simulink model "solar_pv_protected_c07_circuit"  (R2026b)
settings: Solver=VariableStepAuto
model workspace (MAT data in the model file):
  candidate_owner = 'pv_protection_integration_20261023_r01'
  solar_edit_metadata : object (value not decoded)
libraries: fl_lib x149, ee_lib x16, ltc4364demo_lib x3, batteryecm_lib x1, solarprotect_lib x1
(part 9 of 16)

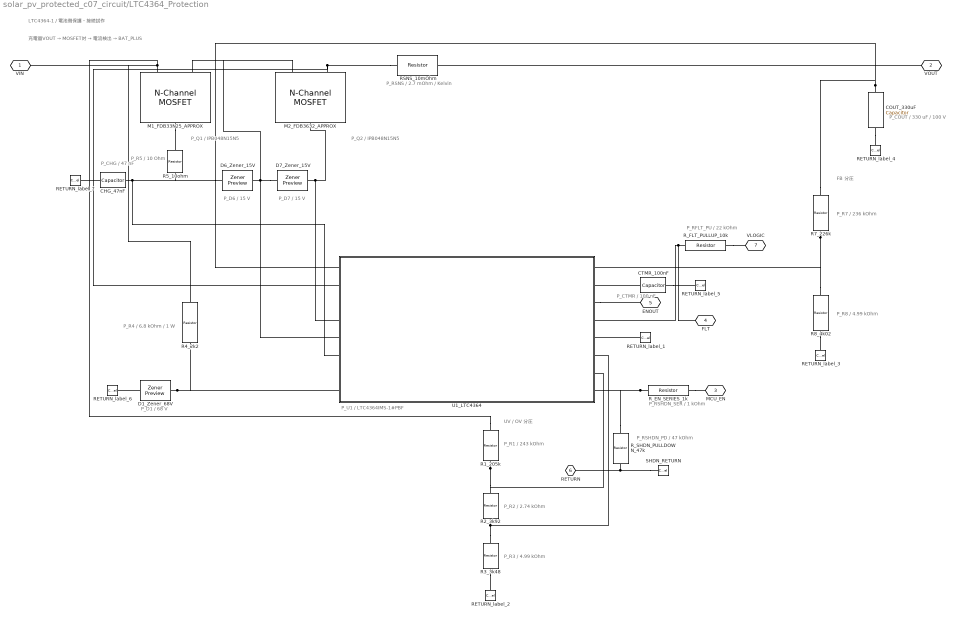
== system solar_pv_protected_c07_circuit/LTC4364_Protection ==
  note: FB 分圧
  note: UV / OV 分圧
  note: 充電器VOUT → MOSFET対 → 電流検出 → BAT_PLUS
  note: LTC4364-1 / 電池側保護・接続試作
  note: P_Q1 / IPB048N15N5
  note: P_Q2 / IPB048N15N5
  note: P_R4 / 6.8 kOhm / 1 W
  note: P_R5 / 10 Ohm
  note: P_RSNS / 2.7 mOhm / Kelvin
  note: P_CHG / 47 nF
  note: P_D6 / 15 V
  note: P_D7 / 15 V
  note: P_COUT / 330 uF / 100 V
  note: P_D1 / 68 V
  note: P_R1 / 243 kOhm
  note: P_R2 / 2.74 kOhm
  note: P_R3 / 4.99 kOhm
  note: P_R7 / 236 kOhm
  note: P_R8 / 4.99 kOhm
  note: P_CTMR / 100 nF
  note: P_RSHDN_SER / 1 kOhm
  note: P_RSHDN_PD / 47 kOhm
  note: P_RFLT_PU / 22 kOhm
  note: P_U1 / LTC4364IMS-1#PBF
  CHG_47nF : fl_lib/Electrical/Electrical Elements/Capacitor  Description=|  c=4.7e-08 F  r=0.01 Ohm  g=1e-10 1/Ohm  i_specify=off  i_priority=None  i=0 A  i_nominal_specify=off  i_nominal_value=1  i_nominal_unit=A  v_specify=off  v_priority=None  v=0 V  v_nominal_specify=off  v_nominal_value=1  v_nominal_unit=V  vc_specify=on  vc_priority=High  vc=0 V  vc_nominal_specify=off  vc_nominal_value=1  vc_nominal_unit=V
      | この回路での名前　　; P_CHG
      | 部品名　　　　　　　; CGA6P3C0G2E473J250AA
      | この回路での役割　　; 保護用MOSFET P_Q1のゲート電圧が立ち上がる速さを調整し、起動時の急な電流を抑える設計に使うコンデンサ。
      | ここでの動き　　　　; 保護ICがP_Q1を駆動する信号P_HGATEと共通GNDの間に47 nFを置き、その充放電によりゲート電圧の変化に時間を持たせる。P_Q1のゲートとソースの間へ直接付けた容量ではなく、起動と故障時の応答の両方に関わる。
      | 
      | 【詳しい働き・仕様・接続・確認の範囲】
      | 部品種別　　　　　　; 保護ゲートスルーレート用コンデンサ
      | 部品分類　　　　　　; 積層セラミックコンデンサ（MLCC）
      | 公称値　　　　　　　; 47 nF
      | 配置目的　　　　　　; HGATE–GND間へ置き、P_Q1起動時のゲート電圧変化と制御応答に関与させる。
      | 意図する動作　　　　; 47 nF。GND基準でありP_Q1のゲート–ソース容量そのものではない。容量変更は突入と故障応答を変える。
      | 端子と接続　　　　　; P P → P_HGATE、N N → GND
      | 部品の耐圧　　　　　; 250 V（既存メーカー資料照合記録の定格。回路全体の適合とは別。）
      | 公称値の公差　　　　; ±5%（既存部品資料の値）
      | 誘電体　　　　　　　; C0G
      | 部品資料の根拠　　　; TDKメーカーMLCC表で該当型番を確認した既存記録。動作時間とPCBでの使用条件は別確認。
      | モデルの範囲　　　　; Simscape標準コンデンサの集中定数表現。材質、DCバイアス、周波数依存ESR/ESL、寿命・温度特性を型番から自動再現するモデルではない。
      | モデル設定　　　　　; c=47 nF、r=10 mΩ、g=100 pS。これらは保存モデルの設定値であり、すべてが実部品の保証値という意味ではない。
      | 損失の扱い　　　　　; 保存モデルの直列抵抗rと実部品の周波数・温度依存ESRは区別する。容量値が一致しても損失・リプル電流・寿命の成立確認にはならない。
      | 確認の範囲　　　　　; 本説明は保存回路の部品情報・端子割当・既存設計意図を整理したもの。今回の説明更新によって新たな動作試験や実機検証を実施した意味ではない。
      | 設計記録　　　　　　; evaluation\component_annotations_20261022_r01\before_graph.json
      | evaluation\component_annotations_20261022_r01\before_metadata.json
      | evaluation\protection_capacitor_integration_20261021_r01\final_delivery\independent_readback\physical_bom.json
      | evaluation\protection_capacitor_integration_20261021_r01\capacitor_review\capacitor_inventory_after_c04.json
      | evaluation\protection_capacitor_integration_20261021_r01\protection_review\component_net_map.json
      | https://product.tdk.com/en/system/files/dam/doc/product/capacitor/ceramic/mlcc/catalog/mlcc_automotive_midvoltage_en.pdf
      | 
      | 【周波数・ノイズと配置の説明】
      | 周波数面の役割　　　; 保護用P_Q1の起動時ゲート電圧が変化する速さを調整し、突入と制御応答に関与する。
      | 対象周波数の目安　　; 主目的は特定周波数のノイズ除去ではなく時間応答の調整。47 nFとICのゲート駆動電流等がゲート電圧の変化速度に関係する。
      | ノイズの発生源　　　; LTC4364がHGATEを充放電するときの電流。ノイズ源に合わせたバイパス容量として選定したという意味ではない。
      | 他のコンデンサとの差; 電源バイパスと異なりHGATE–GND間に接続し、P_Q1のゲート–ソース間の容量そのものでもない。容量変更は起動と故障応答を変える。
      | 周波数説明の範囲　　; スルーレートと突入、保護応答は周辺素子とIC内部動作に依存する。47 nFだけから時間や安全性を保証しない。
      | 周波数説明の根拠　　; Analog Devices：LTC4364-1/LTC4364-2 datasheet
      | https://www.analog.com/media/en/technical-documentation/data-sheets/ltc4364-1-4364-2.pdf
      | 
      | 【この説明欄の略語・記号】
      | 用語1　　　　　　　 ; MLCC：Multilayer Ceramic Capacitor（積層セラミックコンデンサ）。薄いセラミック誘電体と電極を重ねたコンデンサ。対象周波数は容量・実装・寄生成分で変わるため、MLCCという分類だけでは決めない。
      | 用語2　　　　　　　 ; ESR：Equivalent Series Resistance（等価直列抵抗）。コンデンサの損失を直列抵抗で表した量。周波数・温度で変わり、損失とリプル電圧に関係する。
      | 用語3　　　　　　　 ; ESL：Equivalent Series Inductance（等価直列インダクタンス）。端子や電極などの寄生インダクタンスを表す。高い周波数ではバイパス効果を制限する。
      | 用語4　　　　　　　 ; DC：Direct Current（直流）。ここでは直流電源または直流成分。DCバイアスはコンデンサに重なる直流電圧を指す。
      | 用語5　　　　　　　 ; C0G：温度補償系セラミックコンデンサの温度特性記号。英語の頭文字ではなく分類コード。−55〜+125 ℃で容量の温度係数が0±30 ppm/℃の特性を表す。ppmはparts per million（100万分の1）で、30 ppm/℃は1 ℃当たり0.003%に相当する。
      | 用語6　　　　　　　 ; IC：Integrated Circuit（集積回路）。複数の電子素子と機能を小さな半導体チップに集積した部品。
      | 用語7　　　　　　　 ; PWM：Pulse Width Modulation（パルス幅変調）。周期に対するON時間の割合を変えて、スイッチの平均的な電力伝達を調整する方式。
      | 用語8　　　　　　　 ; MOSFET：Metal-Oxide-Semiconductor Field-Effect Transistor（金属・酸化膜・半導体構造の電界効果トランジスタ）。ゲートとソースの電圧でドレインとソースの導通を制御する素子。N-MOSはNチャネル型を表す。
      | 用語9　　　　　　　 ; PCB：Printed Circuit Board（プリント配線板）。部品を実装し、銅配線で接続する基板。
      | 用語10　　　　　　　; GND：Ground（回路の基準電位・電流帰路）。この図の共通基準。保護接地や大地への接続を意味するとは限らない。
      | 用語11　　　　　　　; HGATE/DGATE：LTC4364の二つの外付けMOSFETゲート駆動出力。HGATEは主に電圧・電流制限側のP_Q1、DGATEは理想ダイオード／逆流防止側のP_Q2を駆動する。主電力段の上下PWMとは別の仕組み。
  COUT_330uF : fl_lib/Electrical/Electrical Elements/Capacitor  Description=|  c=330e-6 F  r=0.01 Ohm  g=1e-10 1/Ohm  i_specify=off  i_priority=None  i=0 A  i_nominal_specify=off  i_nominal_value=1  i_nominal_unit=A  v_specify=off  v_priority=None  v=0 V  v_nominal_specify=off  v_nominal_value=1  v_nominal_unit=V  vc_specify=off  vc_priority=High  vc=0 V  vc_nominal_specify=off  vc_nominal_value=1  vc_nominal_unit=V
      | この回路での名前　　; P_COUT
      | 部品名　　　　　　　; 100ZLH330MEFC12.5X35
      | この回路での役割　　; 保護回路を通ったバッテリー側に電荷を蓄え、その場所の電圧・電流の変化を受け止めるためのコンデンサ。
      | ここでの動き　　　　; 保護出力BAT_PLUSと共通GNDの間に330 µFを置く。保護が遮断してもバッテリー側に残るため、保護前のC13〜C16と常に同じ働きをする並列容量としては扱わない。
      | 
      | 【詳しい働き・仕様・接続・確認の範囲】
      | 部品種別　　　　　　; 保護出力側バルクコンデンサ
      | 部品分類　　　　　　; アルミ電解コンデンサ（有極性）
      | 公称値　　　　　　　; 330 µF
      | 配置目的　　　　　　; BAT_PLUS–GND間へ配置し、保護回路下流側の局所的な電荷を受け持つ。
      | 意図する動作　　　　; 上流VOUTのC13〜C16とは保護OFF時に別ノードとなり、同じ目的の重複部品ではない。330 µFの実効容量・リプル・熱の適合は別確認。
      | 端子と接続　　　　　; P P → BAT_PLUS、N N → GND
      | 部品の耐圧　　　　　; 100 V（既存メーカー資料照合記録の定格。回路全体の適合とは別。）
      | 公称値の公差　　　　; ±20%（既存部品資料の値）
      | 部品資料の根拠　　　; Rubycon ZLHメーカー表の100 V・330 µF・12.5×35 mmと品番構成に基づく既存照合記録。43 mΩは100 kHzインピーダンスの上限であり、全周波数の一定ESRではない。
      | モデルの範囲　　　　; Simscape標準コンデンサの集中定数表現。材質、DCバイアス、周波数依存ESR/ESL、寿命・温度特性を型番から自動再現するモデルではない。
      | モデル設定　　　　　; c=330 µF、r=10 mΩ、g=100 pS。これらは保存モデルの設定値であり、すべてが実部品の保証値という意味ではない。
      | 損失の扱い　　　　　; 保存モデルの直列抵抗rと実部品の周波数・温度依存ESRは区別する。容量値が一致しても損失・リプル電流・寿命の成立確認にはならない。
      | 確認の範囲　　　　　; 本説明は保存回路の部品情報・端子割当・既存設計意図を整理したもの。今回の説明更新によって新たな動作試験や実機検証を実施した意味ではない。
      | 設計記録　　　　　　; evaluation\component_annotations_20261022_r01\before_graph.json
      | evaluation\component_annotations_20261022_r01\before_metadata.json
      | evaluation\protection_capacitor_integration_20261021_r01\final_delivery\independent_readback\physical_bom.json
      | evaluation\protection_capacitor_integration_20261021_r01\capacitor_review\capacitor_inventory_after_c04.json
      | evaluation\protection_capacitor_integration_20261021_r01\protection_review\component_net_map.json
      | https://www.rubycon.co.jp/wp-content/uploads/catalog-aluminum/ZLH.pdf
      | 
      | 【周波数・ノイズと配置の説明】
      | 周波数面の役割　　　; 保護回路の下流BAT_PLUS側に局所的な電荷を蓄える。
      | 対象周波数の目安　　; 起動/遮断/負荷変化の過渡と、通電時に上流から届くリプルが対象。具体的な有効帯域は回路と実装に依存する。
      | ノイズの発生源　　　; 保護MOSFETをオン・オフする過渡、配線を通じたバッテリー電流変化、保護が導通中の上流降圧回路のリプル。
      | 他のコンデンサとの差; C13/C14の上流VOUT側と異なり、遮断中もBAT_PLUS側に残る330 µF電解。上流の大容量と単純に並列合算できない。
      | 周波数説明の範囲　　; 狙うノイズの周波数と、この部品が実装後に有効な周波数範囲は別である。実効容量、等価直列抵抗、等価直列インダクタンス、配線を含む自己共振で変わるため、型番名や公称容量だけから有効帯域の上限を断定しない。
      | 周波数説明の根拠　　; Analog Devices：LTC4364-1/LTC4364-2 datasheet
      | https://www.analog.com/media/en/technical-documentation/data-sheets/ltc4364-1-4364-2.pdf
      | 村田製作所：コンデンサのインピーダンス・ESRと周波数の関係
      | https://article.murata.com/en-global/article/impedance-esr-frequency-characteristics-in-capacitors
      | 
      | 【この説明欄の略語・記号】
      | 用語1　　　　　　　 ; ESR：Equivalent Series Resistance（等価直列抵抗）。コンデンサの損失を直列抵抗で表した量。周波数・温度で変わり、損失とリプル電圧に関係する。
      | 用語2　　　　　　　 ; ESL：Equivalent Series Inductance（等価直列インダクタンス）。端子や電極などの寄生インダクタンスを表す。高い周波数ではバイパス効果を制限する。
      | 用語3　　　　　　　 ; DC：Direct Current（直流）。ここでは直流電源または直流成分。DCバイアスはコンデンサに重なる直流電圧を指す。
      | 用語4　　　　　　　 ; MOSFET：Metal-Oxide-Semiconductor Field-Effect Transistor（金属・酸化膜・半導体構造の電界効果トランジスタ）。ゲートとソースの電圧でドレインとソースの導通を制御する素子。N-MOSはNチャネル型を表す。
      | 用語5　　　　　　　 ; GND：Ground（回路の基準電位・電流帰路）。この図の共通基準。保護接地や大地への接続を意味するとは限らない。
      | 用語6　　　　　　　 ; VIN/VOUT：入力電圧・出力電圧を表す端子／ネット名。INは入力、OUTは出力。電源変換器の電力端子なのか、検出用端子なのかは対象部品によって異なるため、端子と接続の説明に従う。
  CTMR_100nF : fl_lib/Electrical/Electrical Elements/Capacitor  Description=|  c=1e-07 F  r=0.01 Ohm  g=1e-10 1/Ohm  i_specify=off  i_priority=None  i=0 A  i_nominal_specify=off  i_nominal_value=1  i_nominal_unit=A  v_specify=off  v_priority=None  v=0 V  v_nominal_specify=off  v_nominal_value=1  v_nominal_unit=V  vc_specify=on  vc_priority=High  vc=0 V  vc_nominal_specify=off  vc_nominal_value=1  vc_nominal_unit=V
      | この回路での名前　　; P_CTMR
      | 部品名　　　　　　　; CGA5L2C0G1H104J160AE
      | この回路での役割　　; 保護ICが異常の継続時間を判断し、遮断へ移るタイミングを決めるためのコンデンサ。
      | ここでの動き　　　　; 保護ICの時間設定信号P_TMRと共通GNDの間に100 nFを置き、内部電流による充放電を時間の判断に使う。遮断までの時間は容量だけでなく、故障状態やIC内部の電流・判定電圧にも依存する。
      | 
      | 【詳しい働き・仕様・接続・確認の範囲】
      | 部品種別　　　　　　; 保護故障タイマ用コンデンサ
      | 部品分類　　　　　　; 積層セラミックコンデンサ（MLCC）
      | 公称値　　　　　　　; 100 nF
      | 配置目的　　　　　　; TMR–GND間に置き、故障継続時間の積算・遮断タイミングへ関与させる。
      | 意図する動作　　　　; 100 nF。タイマ電流と比較しきい値にも依存し、公称容量だけで遮断時間は一意に保証されない。
      | 端子と接続　　　　　; P P → P_TMR、N N → GND
      | 部品の耐圧　　　　　; 50 V（既存メーカー資料照合記録の定格。回路全体の適合とは別。）
      | 公称値の公差　　　　; ±5%（既存部品資料の値）
      | 誘電体　　　　　　　; C0G
      | 部品資料の根拠　　　; TDKメーカーMLCC表で該当型番を確認した既存記録。動作時間とPCBでの使用条件は別確認。
      | モデルの範囲　　　　; Simscape標準コンデンサの集中定数表現。材質、DCバイアス、周波数依存ESR/ESL、寿命・温度特性を型番から自動再現するモデルではない。
      | モデル設定　　　　　; c=100 nF、r=10 mΩ、g=100 pS。これらは保存モデルの設定値であり、すべてが実部品の保証値という意味ではない。
      | 損失の扱い　　　　　; 保存モデルの直列抵抗rと実部品の周波数・温度依存ESRは区別する。容量値が一致しても損失・リプル電流・寿命の成立確認にはならない。
      | 確認の範囲　　　　　; 本説明は保存回路の部品情報・端子割当・既存設計意図を整理したもの。今回の説明更新によって新たな動作試験や実機検証を実施した意味ではない。
      | 設計記録　　　　　　; evaluation\component_annotations_20261022_r01\before_graph.json
      | evaluation\component_annotations_20261022_r01\before_metadata.json
      | evaluation\protection_capacitor_integration_20261021_r01\final_delivery\independent_readback\physical_bom.json
      | evaluation\protection_capacitor_integration_20261021_r01\capacitor_review\capacitor_inventory_after_c04.json
      | evaluation\protection_capacitor_integration_20261021_r01\protection_review\component_net_map.json
      | https://product.tdk.com/system/files/dam/doc/product/capacitor/ceramic/mlcc/catalog/mlcc_automotive_soft_en.pdf
      | 
      | 【周波数・ノイズと配置の説明】
      | 周波数面の役割　　　; 故障がどれだけ継続したかを電荷として積算し、遮断までの時間に関与するタイマ容量。
      | 対象周波数の目安　　; 主目的はノイズの周波数選別ではない。容量、IC内部の充放電電流、比較しきい値から時間が決まるため、「100 nFの高周波ノイズ用」とは説明しない。
      | ノイズの発生源　　　; 想定する入力はLTC4364の故障状態に応じたタイマ充放電。測定したノイズ周波数をこの部品へ割り当ててはいない。
      | 他のコンデンサとの差; 同じ100 nFのC17/C36等は電源バイパス。本品は時間設定であり、部品種が同じでも役割は異なる。
      | 周波数説明の範囲　　; 遮断時間は型番の内部電流・しきい値、故障条件、初期状態も含めて評価する。公称容量だけで保証しない。
      | 周波数説明の根拠　　; Analog Devices：LTC4364-1/LTC4364-2 datasheet
      | https://www.analog.com/media/en/technical-documentation/data-sheets/ltc4364-1-4364-2.pdf
      | 
      | 【この説明欄の略語・記号】
      | 用語1　　　　　　　 ; MLCC：Multilayer Ceramic Capacitor（積層セラミックコンデンサ）。薄いセラミック誘電体と電極を重ねたコンデンサ。対象周波数は容量・実装・寄生成分で変わるため、MLCCという分類だけでは決めない。
      | 用語2　　　　　　　 ; ESR：Equivalent Series Resistance（等価直列抵抗）。コンデンサの損失を直列抵抗で表した量。周波数・温度で変わり、損失とリプル電圧に関係する。
      | 用語3　　　　　　　 ; ESL：Equivalent Series Inductance（等価直列インダクタンス）。端子や電極などの寄生インダクタンスを表す。高い周波数ではバイパス効果を制限する。
      | 用語4　　　　　　　 ; DC：Direct Current（直流）。ここでは直流電源または直流成分。DCバイアスはコンデンサに重なる直流電圧を指す。
      | 用語5　　　　　　　 ; C0G：温度補償系セラミックコンデンサの温度特性記号。英語の頭文字ではなく分類コード。−55〜+125 ℃で容量の温度係数が0±30 ppm/℃の特性を表す。ppmはparts per million（100万分の1）で、30 ppm/℃は1 ℃当たり0.003%に相当する。
      | 用語6　　　　　　　 ; IC：Integrated Circuit（集積回路）。複数の電子素子と機能を小さな半導体チップに集積した部品。
      | 用語7　　　　　　　 ; PCB：Printed Circuit Board（プリント配線板）。部品を実装し、銅配線で接続する基板。
      | 用語8　　　　　　　 ; GND：Ground（回路の基準電位・電流帰路）。この図の共通基準。保護接地や大地への接続を意味するとは限らない。
      | 用語9　　　　　　　 ; TMR：Timer（時間設定端子）。LTC4364では外付けコンデンサにより故障継続時間の判定などに関係する時間を設定する。
  D1_Zener_68V : ltc4364demo_lib/Zener Preview  Description=|  Vz=68 V  Rz=5 Ohm  Vf=0.7 V  Rf=1 Ohm  i_specify=off  i_priority=None  i=0 A  i_nominal_specify=off  i_nominal_value=1  i_nominal_unit=A
      | この回路での名前　　; P_D1
      | 部品名　　　　　　　; CMZ5945B TR13 PBFREE
      | この回路での役割　　; 保護IC P_U1の電源電圧が上がりすぎるのを抑えるダイオード。
      | ここでの動き　　　　; 保護ICの電源とGNDの間に接続し、電圧が上がったときに電流を逃がす。直列抵抗P_R4と組み合わせて使う。
      | 
      | 【詳しい働き・仕様・接続・確認の範囲】
      | 部品種別　　　　　　; 保護IC電源クランプ・ツェナー
      | 公称値　　　　　　　; 68 V
      | 配置目的　　　　　　; P_VCC–GND間でLTC4364の電源電圧上昇を抑える。
      | 意図する動作　　　　; 公称68 V。P_R4と組み合わせる。クランプ公差・電流依存・持続損失・PCB放熱の成立は別確認。
      | 端子と接続　　　　　; A A → GND、K K → P_VCC
      | 部品資料の根拠　　　; Central Semiconductor公式製品情報のCMZ5945B TR13と、鉛フリー接尾辞PBFREEの既存確認記録。
      | モデルの範囲　　　　; Simscapeダイオード素子による近似。順方向損失、漏れ、温度依存、逆回復・接合容量の型番固有特性を完全に再現するものではない。
      | モデル設定　　　　　; Vf=700 mV、Vz=68 V。これらは保存モデルの設定値であり、すべてが実部品の保証値という意味ではない。
      | 確認の範囲　　　　　; 本説明は保存回路の部品情報・端子割当・既存設計意図を整理したもの。今回の説明更新によって新たな動作試験や実機検証を実施した意味ではない。
      | 設計記録　　　　　　; evaluation\component_annotations_20261022_r01\before_graph.json
      | evaluation\component_annotations_20261022_r01\before_metadata.json
      | evaluation\protection_capacitor_integration_20261021_r01\final_delivery\independent_readback\physical_bom.json
      | evaluation\protection_capacitor_integration_20261021_r01\protection_review\component_net_map.json
      | 
      | 【この説明欄の略語・記号】
      | 用語1　　　　　　　 ; IC：Integrated Circuit（集積回路）。複数の電子素子と機能を小さな半導体チップに集積した部品。
      | 用語2　　　　　　　 ; MOSFET：Metal-Oxide-Semiconductor Field-Effect Transistor（金属・酸化膜・半導体構造の電界効果トランジスタ）。ゲートとソースの電圧でドレインとソースの導通を制御する素子。N-MOSはNチャネル型を表す。
      | 用語3　　　　　　　 ; Vf：Forward Voltage（順方向電圧）。ダイオードが順方向に電流を流すときの電圧降下。電流・温度で変わる。
      | 用語4　　　　　　　 ; Vz：Zener Voltage（ツェナー電圧）。ツェナーダイオードの逆方向での電圧制限に関係する値。
      | 用語5　　　　　　　 ; PCB：Printed Circuit Board（プリント配線板）。部品を実装し、銅配線で接続する基板。
      | 用語6　　　　　　　 ; GND：Ground（回路の基準電位・電流帰路）。この図の共通基準。保護接地や大地への接続を意味するとは限らない。
      | 用語7　　　　　　　 ; VCC/VDD/VEE/VS：ICの電源端子名。文字の歴史的な由来を現在の接続機能へ当てはめない。現回路のVEEはU8/U10では浮動基準SW、U9ではGND。各電圧・基準は端子と接続を参照する。
      | 用語8　　　　　　　 ; SW：Switching Node（スイッチング点）。主電力段の上下MOSFETとL1がつながる、電圧が高速に切り替わる点。GNDとは別電位。
  D6_Zener_15V : ltc4364demo_lib/Zener Preview  Description=|  Vz=15 V  Rz=5 Ohm  Vf=0.7 V  Rf=1 Ohm  i_specify=off  i_priority=None  i=0 A  i_nominal_specify=off  i_nominal_value=1  i_nominal_unit=A
      | この回路での名前　　; P_D6
      | 部品名　　　　　　　; DDZ9702T
      | この回路での役割　　; 保護用MOSFET P_Q1を駆動する電圧が、ソースに対して高くなりすぎるのを抑えるダイオード。
      | ここでの動き　　　　; 保護ICのゲート駆動出力HGATEと、P_Q1/P_Q2共通のソース点の間に置く。共通GNDに対する電圧を抑える部品ではない。
      | 
      | 【詳しい働き・仕様・接続・確認の範囲】
      | 部品種別　　　　　　; HGATE–共通ソース間ツェナー
      | 公称値　　　　　　　; 15 V
      | 配置目的　　　　　　; HGATEとP_SOURCE間でP_Q1側のゲート電圧上昇を抑える。
      | 意図する動作　　　　; 公称15 V。P_SOURCEはGNDではない。P_R5よりIC側に配置されたクランプ。
      | 端子と接続　　　　　; A A → P_SOURCE、K K → P_HGATE
      | 部品資料の根拠　　　; Diodes Incorporated DDZ96xxT/DDZ97xxTデータシートに公称15 VのDDZ9702Tを確認した既存記録。梱包接尾辞とパルス電力の適合は未確定。
      | モデルの範囲　　　　; Simscapeダイオード素子による近似。順方向損失、漏れ、温度依存、逆回復・接合容量の型番固有特性を完全に再現するものではない。
      | モデル設定　　　　　; Vf=700 mV、Vz=15 V。これらは保存モデルの設定値であり、すべてが実部品の保証値という意味ではない。
      | 確認の範囲　　　　　; 本説明は保存回路の部品情報・端子割当・既存設計意図を整理したもの。今回の説明更新によって新たな動作試験や実機検証を実施した意味ではない。
      | 設計記録　　　　　　; evaluation\component_annotations_20261022_r01\before_graph.json
      | evaluation\component_annotations_20261022_r01\before_metadata.json
      | evaluation\protection_capacitor_integration_20261021_r01\final_delivery\independent_readback\physical_bom.json
      | evaluation\protection_capacitor_integration_20261021_r01\protection_review\component_net_map.json
      | 
      | 【この説明欄の略語・記号】
      | 用語1　　　　　　　 ; IC：Integrated Circuit（集積回路）。複数の電子素子と機能を小さな半導体チップに集積した部品。
      | 用語2　　　　　　　 ; PWM：Pulse Width Modulation（パルス幅変調）。周期に対するON時間の割合を変えて、スイッチの平均的な電力伝達を調整する方式。
      | 用語3　　　　　　　 ; MOSFET：Metal-Oxide-Semiconductor Field-Effect Transistor（金属・酸化膜・半導体構造の電界効果トランジスタ）。ゲートとソースの電圧でドレインとソースの導通を制御する素子。N-MOSはNチャネル型を表す。
      | 用語4　　　　　　　 ; Vf：Forward Voltage（順方向電圧）。ダイオードが順方向に電流を流すときの電圧降下。電流・温度で変わる。
      | 用語5　　　　　　　 ; Vz：Zener Voltage（ツェナー電圧）。ツェナーダイオードの逆方向での電圧制限に関係する値。
      | 用語6　　　　　　　 ; GND：Ground（回路の基準電位・電流帰路）。この図の共通基準。保護接地や大地への接続を意味するとは限らない。
      | 用語7　　　　　　　 ; HGATE/DGATE：LTC4364の二つの外付けMOSFETゲート駆動出力。HGATEは主に電圧・電流制限側のP_Q1、DGATEは理想ダイオード／逆流防止側のP_Q2を駆動する。主電力段の上下PWMとは別の仕組み。
  D7_Zener_15V : ltc4364demo_lib/Zener Preview  Description=|  Vz=15 V  Rz=5 Ohm  Vf=0.7 V  Rf=1 Ohm  i_specify=off  i_priority=None  i=0 A  i_nominal_specify=off  i_nominal_value=1  i_nominal_unit=A
      | この回路での名前　　; P_D7
      | 部品名　　　　　　　; DDZ9702T
      | この回路での役割　　; 逆流防止用MOSFET P_Q2のゲート電圧が、ソースに対して高くなりすぎるのを抑えるダイオード。
      | ここでの動き　　　　; 保護ICのゲート駆動出力DGATEと、P_Q1/P_Q2共通のソース点の間に置く。
      | 
      | 【詳しい働き・仕様・接続・確認の範囲】
      | 部品種別　　　　　　; DGATE–共通ソース間ツェナー
      | 公称値　　　　　　　; 15 V
      | 配置目的　　　　　　; DGATEとP_SOURCE間でP_Q2のゲート電圧上昇を抑える。
      | 意図する動作　　　　; 公称15 V。動的クランプとパルス電力は未適合確認。
      | 端子と接続　　　　　; A A → P_SOURCE、K K → P_DGATE
      | 部品資料の根拠　　　; Diodes Incorporated DDZ96xxT/DDZ97xxTデータシートに公称15 VのDDZ9702Tを確認した既存記録。梱包接尾辞とパルス電力の適合は未確定。
      | モデルの範囲　　　　; Simscapeダイオード素子による近似。順方向損失、漏れ、温度依存、逆回復・接合容量の型番固有特性を完全に再現するものではない。
      | モデル設定　　　　　; Vf=700 mV、Vz=15 V。これらは保存モデルの設定値であり、すべてが実部品の保証値という意味ではない。
      | 確認の範囲　　　　　; 本説明は保存回路の部品情報・端子割当・既存設計意図を整理したもの。今回の説明更新によって新たな動作試験や実機検証を実施した意味ではない。
      | 設計記録　　　　　　; evaluation\component_annotations_20261022_r01\before_graph.json
      | evaluation\component_annotations_20261022_r01\before_metadata.json
      | evaluation\protection_capacitor_integration_20261021_r01\final_delivery\independent_readback\physical_bom.json
      | evaluation\protection_capacitor_integration_20261021_r01\protection_review\component_net_map.json
      | 
      | 【この説明欄の略語・記号】
      | 用語1　　　　　　　 ; PWM：Pulse Width Modulation（パルス幅変調）。周期に対するON時間の割合を変えて、スイッチの平均的な電力伝達を調整する方式。
      | 用語2　　　　　　　 ; MOSFET：Metal-Oxide-Semiconductor Field-Effect Transistor（金属・酸化膜・半導体構造の電界効果トランジスタ）。ゲートとソースの電圧でドレインとソースの導通を制御する素子。N-MOSはNチャネル型を表す。
      | 用語3　　　　　　　 ; Vf：Forward Voltage（順方向電圧）。ダイオードが順方向に電流を流すときの電圧降下。電流・温度で変わる。
      | 用語4　　　　　　　 ; Vz：Zener Voltage（ツェナー電圧）。ツェナーダイオードの逆方向での電圧制限に関係する値。
      | 用語5　　　　　　　 ; HGATE/DGATE：LTC4364の二つの外付けMOSFETゲート駆動出力。HGATEは主に電圧・電流制限側のP_Q1、DGATEは理想ダイオード／逆流防止側のP_Q2を駆動する。主電力段の上下PWMとは別の仕組み。
  M1_FDB33N25_APPROX : ee_lib/Semiconductors & Converters/N-Channel MOSFET  Description=|  paramTerminal=ee.enum.mosfet.numberOfTerminals.three  parameterization=ee.enum.mosfet.parameterization.datasheet  Beta=5.0 A/V^2  Rds=0.0048 Ohm  Id=4 A  Vgs=10 V  Vth=4.1 V  Vth0=1.7 V  lam=0 1/V  gamma_vth=0.5 V^(1/2)  phib=0.5 V  Vth1=1.9071 V  Vbs1=-1 V  Vth2=2.066 V  Vbs2=-2 V  Tmeas=25 degC  Vgs_vec=[-1, -.5, 2, 3, 4, 5] V  Vds_vec=[0, 2, 4, 8, 12, 16, 20] V  Vbs_vec=[0, -4, -6, -12] V  T_vec=[25, 125] degC  Vth_vec=[.4, 1.2, 1.4, 1.45] V  Vth_mat=[.4, .35; 1.2, 1.15; 1.4, 1.35; 1.45, 1.4] V  Ids_mat=[0, 0, 0, 0, 0, 0, 0; 0, 0, 0, 0, 0, 0, 0; 0, .003, .0038, .0043, .0046, .0048, .0049; 0, .0055, .008, .009, .0095, .01, .0101; 0, .0115, .016, .018, .019, .0195, .02; 0, .0152, .0225, .0265, .028, .0295, .03] A  Ids_mat0=[0, 0, 0, 0, 0, 0, 0; 0, 0, 0, 0, 0, 0, 0; 0, .003, .0038, .0043, .0046, .0048, .0049; 0, .0055, .008, .009, .0095, .01, .0101; 0, .0115, .016, .018, .019, .0195, .02; 0, .0152, .0225, .0265, .028, .0295, .03] A  Ids_mat_3D=zeros(6, 7, 2) A  Ids_mat_3D0=zeros(6, 7, 2) A  IV_table_symmetry=ee.enum.mosfet.symmetricNIV.no  RS=0.0001 Ohm  RD=0.0001 Ohm  RB=0.001 Ohm  LeadRs=0 Ohm  LeadRd=0 Ohm  LeadRg=25 Ohm  LeadRb=0 Ohm  LS=0 nH  LD=0 nH  LG=0 nH  LB=0 nH  C_param=ee.enum.mosfet.capacitanceParam.fixedciss  C_GS=270 pF  C_GD=80 pF  C_GB=0 pF  C_DS=0 pF  C_iss=290e-12 F  C_rss=13e-12 F  C_oss=1400e-12 F  C_iss_vec=[720, 700, 590, 470, 390, 310] pF  C_rss_vec=[450, 400, 300, 190, 95, 55] pF  C_oss_vec=[900, 810, 690, 420, 270, 170] pF  C_GS_vec=[270, 300, 290, 280, 295, 255] pF  C_GD_vec=[450, 400, 300, 190, 95, 55] pF  C_GB_vec=[270, 300, 290, 280, 295, 255] pF  C_Vgs_vec=0 V  C_DS_vec=[450, 410, 390, 230, 175, 115] pF  C_Vds_vec=[.1, .3, 1, 3, 10, 30] V  V_GS_for_cap_data=0 V  charge_linearity_param=ee.enum.mosfet.cgdLinearity.constant  C_OX=200 pF  V_C_OX=-0.5 V  charge_linearity_param_vgb=ee.enum.mosfet.cgbLinearity.instantly  charge_linearity_param_with_vgb=ee.enum.mosfet.cgbLinearityWithSeparateCgb.instantly  Di_param=ee.enum.mosfet.diodeParam.exponential  IsDiode=1e-9 A  Vbi=0.6 V  n=1.5  Cj0Diode=0 pF  TT=0 s  Tmeas_dio=25 degC  TableTypeNoT=ee.enum.mosfet.tableType.IfMat  TableType=ee.enum.diode.tableType.IfMat  IfVec=[.07, .12, .19, 1.75, 4.24, 7.32, 11.2] A  IfMat=[.07, .12, .19, 1.75, 4.24, 7.32, 11.2; .16, .3, .72, 2.14, 4.02, 6.35, 9.12] A  VfVecV=[.9, 1.15, 1.25, 1.5, 1.75, 2.17, 2.6, 2.85] V  VfMatV=[.9, 1.15, 1.25, 1.5, 1.75, 2.17, 2.6, 2.85; .58, .68, .75, 1.1, 1.38, 1.77, 2.27, 2.7] V  TjVec=[25, 125] degC  VfVec=[.5, .7, .9, 1.3, 1.7, 2.1, 2.5] V  IfVecV=[.1, .2, .5, 1, 2, 4, 7, 10] A  diode_Goff=1e-12 1/Ohm  prmDatasheet=ee.enum.temperatureParameterization.none  prmEquCoeff=ee.enum.temperatureParameterization.none  dVth_dT=-6 mV/K  dVth0_dT=-6 mV/K  Rds_T2=0.037 Ohm  BEXDatasheet=-1.5  BEXEquCoeff=-1.5  etaisDatasheet=3  etaisEquCoeff=3  Tmeas2=125 degC  etaisTabulated=3  TdeviceDatasheet=25 degC  TdeviceEquCoeff=25 degC  TdeviceTabulated=25 degC  i_g_specify=off  i_g_priority=None  i_g=0 A  i_g_nominal_specify=off  i_g_nominal_value=1  i_g_nominal_unit=A  i_d_specify=off  i_d_priority=None  i_d=0 A  i_d_nominal_specify=off  i_d_nominal_value=1  i_d_nominal_unit=A  i_b_specify=off  i_b_priority=None  i_b=0 A  i_b_nominal_specify=off  i_b_nominal_value=1  i_b_nominal_unit=A  voltage_gs_specify=off  voltage_gs_priority=None  voltage_gs=0 V  voltage_gs_nominal_specify=off  voltage_gs_nominal_value=1  voltage_gs_nominal_unit=V  voltage_ds_specify=off  voltage_ds_priority=None  voltage_ds=0 V  voltage_ds_nominal_specify=off  voltage_ds_nominal_value=1  voltage_ds_nominal_unit=V  voltage_bs_specify=off  voltage_bs_priority=None  voltage_bs=0 V  voltage_bs_nominal_specify=off  voltage_bs_nominal_value=1  voltage_bs_nominal_unit=V  v_Cgs_specify=off  v_Cgs_priority=High  v_Cgs=0 V  v_Cgs_nominal_specify=off  v_Cgs_nominal_value=1  v_Cgs_nominal_unit=V  v_Cds_specify=off  v_Cds_priority=High  v_Cds=0 V  v_Cds_nominal_specify=off  v_Cds_nominal_value=1  v_Cds_nominal_unit=V  v_Cbs_specify=off  v_Cbs_priority=High  v_Cbs=0 V  v_Cbs_nominal_specify=off  v_Cbs_nominal_value=1  v_Cbs_nominal_unit=V  thermal_network_parameterization=ee.enum.thermalNetworkTopology.junctionCase  Rth=[0, 10] K/W  Rth_Cauer=[1, 3, 10] K/W  Rth_Foster=[.08, .14, .22, .16] K/W  thermal_mass_parameterization=ee.enum.thermalNetwork.timeconstant  thermal_mass=[0, 1] J/K  thermal_mass_Cauer=[.1, .3, 1] J/K  thermal_mass_Foster=[.001, .005, .05, .5] J/K  thermal_time_constant=[0, 10] s  thermal_time_constant_Cauer=[1, 3, 10] s  thermal_time_constant_Foster=[7e-05, .0007, .01, .08] s  thermal_mass_initial_temperatures=[25, 25] degC  thermal_mass_initial_temperatures_Cauer=[25, 25, 25] degC  Tvec_initial_Foster=[25, 25, 25, 25] degC  betaref=18 A/V^2  Vfbref=-1.1 V  gamma=3.5 V^(1/2)  phib2ref=1 V  thesatref=0.4 1/V  alpha=0  Vp=5e-2 V  thesrref=0 1/V  m=8  Tref=25 degC  Rsref=2e-3 Ohm  Rdref=0.17 Ohm  Rgref=8.4 Ohm  Rbref=2e-3 Ohm  Cox=1500 pF  Cgso=100 pF  Cgdo=14 pF  Isref=5.2e-13 A  Cj0=480 pF  Tprm=ee.enum.temperatureParameterization.none  etabet=1.3  Stvfb=5e-4 V/K  Stphib=-8.5e-4 V/K  etasat=1.04  etasr=0.65  etar=0.95  etais=3  Tsim=25 degC  Ig_specify=off  Ig_priority=None  Ig=0 A  Ig_nominal_specify=off  Ig_nominal_value=1  Ig_nominal_unit=nA  Ids_specify=off  Ids_priority=None  Ids=0 A  Ids_nominal_specify=off  Ids_nominal_value=1  Ids_nominal_unit=A  Ib_specify=off  Ib_priority=None  Ib=0 A  Ib_nominal_specify=off  Ib_nominal_value=1  Ib_nominal_unit=uA  V_gs_specify=off  V_gs_priority=None  V_gs=0 V  V_gs_nominal_specify=off  V_gs_nominal_value=1  V_gs_nominal_unit=V  V_ds_specify=off  V_ds_priority=None  V_ds=0 V  V_ds_nominal_specify=off  V_ds_nominal_value=1  V_ds_nominal_unit=V  V_bs_specify=off  V_bs_priority=None  V_bs=0 V  V_bs_nominal_specify=off  V_bs_nominal_value=1  V_bs_nominal_unit=V  QGoverCox_specify=off  QGoverCox_priority=None  QGoverCox=0 V  QGoverCox_nominal_specify=off  QGoverCox_nominal_value=1  QGoverCox_nominal_unit=V  QDoverCox_specify=off  QDoverCox_priority=None  QDoverCox=0 V  QDoverCox_nominal_specify=off  QDoverCox_nominal_value=1  QDoverCox_nominal_unit=V  QBoverCox_specify=off  QBoverCox_priority=None  QBoverCox=0 V  QBoverCox_nominal_specify=off  QBoverCox_nominal_value=1  QBoverCox_nominal_unit=V  T0=[25, 25] degC  T0_Cauer=[25, 25, 25] degC
      | この回路での名前　　; P_Q1
      | 部品名　　　　　　　; IPB048N15N5LFATMA1
      | この回路での役割　　; 電池へ流す充電電流を通し、起動時や異常時には電流・電圧を制限するための保護用MOSFET。
      | ここでの動き　　　　; 保護IC P_U1の指令で、十分にONする通常状態と、導通を絞る制限状態やOFF状態を使い分ける。主電力段Q1/Q2のような周期的な充電制御スイッチではない。
      | 
      | 【詳しい働き・仕様・接続・確認の範囲】
      | 識別の補足　　　　　; P_Q1。「P」はProtection（保護回路）の区分、「Q1」はその中の素子番号。
      | 
      | 配置目的　　　　　　; 充電器から蓄電池へ向かう電力経路を開閉し、起動時や異常時には流れる電流・出力電圧を制限するために置く。
      | 接続　　　　　　　　; ドレインは充電器出力VOUT、ソースはP_Q2と共通のP_SOURCEへ接続する。ゲートはLTC4364のHGATEから外付け10 Ωを介して駆動する。P_SOURCEは2個のMOSFETの共通ソース点であり、GNDではない。
      | 制御担当　　　　　　; LTC4364のHGATE側。主電力段Q1/Q2のような相補PWM駆動は行わない。
      | 
      | 正常時の想定動作　　; 十分にONにして充電電流を通す。このときの電圧降下と発熱を小さくするため、低いON抵抗を利用する。
      | 起動時の想定動作　　; ゲート電圧を徐々に上げ、急激な通電を抑えながら充電経路を導通させる。
      | 異常時の想定動作　　; LTC4364がP_Q1のゲートを調整し、導通を絞って電流や出力電圧を制限する。異常が続いた場合はタイマによって遮断する。運転中の出力過電圧制限はFB端子側の機能であり、OV端子の起動禁止判定とは区別する。
      | 停止時の想定動作　　; SHDNによる停止やラッチ故障時にはゲートを下げる。逆流防止の主担当はP_Q2であり、逆流時にP_Q1も必ずOFFになるとは限らない。
      | 
      | メーカーの用途　　　; メーカーはこの品種をホットスワップ（通電状態での接続）や電子ヒューズ用途向けと説明し、広いSOAを特徴としている。
      | 選定理由　　　　　　; P_Q1は異常時に単純なON/OFFだけでなく、電流を流しながら素子両端に電圧を受け持つ使い方をする。このような途中まで導通させる動作を考慮した品種であることが、保護用の直列MOSFETとして選ぶ根拠になる。ただし、実際の電圧・電流・時間・温度がSOA内に入るかは別途確認する。
      | 
      | 部品種別　　　　　　; NチャネルMOSFET（保護経路用）。
      | 部品分類　　　　　　; 150 V linear-mode MOSFET（リニア動作を考慮した品種）。
      | メーカー　　　　　　; Infineon。
      | 部品名の補足　　　　; IPB048N15N5LFATMA1（基本型番：IPB048N15N5LF）。
      | 採用状態　　　　　　; 現モデルへ割り当てた実部品候補。実部品としての全条件での成立確認は未完了。
      | 
      | 耐圧　　　　　　　　; ドレイン－ソース間150 V。端子間電圧の定格であり、この値だけで回路全体の安全性は判断しない。
      | 導通時抵抗　　　　　; 最大4.8 mΩ、代表3.9 mΩ。測定条件は接合温度25 ℃、ゲート－ソース電圧10 V、ドレイン電流100 A。
      | 内部ゲート抵抗　　　; 代表25 Ω、最大38 Ω。メーカーの設計規定値であり、出荷時の全数測定値ではない。
      | 総ゲート電荷　　　　; 代表84 nC。VDD=75 V、ID=60 A、VGS=0→10 Vの条件。
      | 
      | モデル抵抗近似　　　; 内部ゲート抵抗の代表値25 Ωを、SimscapeのGate lead resistance（LeadRg）にまとめて近似している。外付け抵抗を25 Ω追加した意味でも、パッケージのリードだけが25 Ωという意味でもない。
      | モデル容量近似　　　; VGS=0 V、VDS=75 V、1 MHzでの代表容量Ciss=290 pF、Coss=1400 pF、Crss=13 pFを固定値として使う。電圧で変化する容量や総ゲート電荷84 nCを再現したモデルではない。
      | モデル導通特性　　　; 現在のモデルの校正用電流パラメータIdは4 Aであり、ON抵抗のメーカー測定条件100 Aと一致していない。4 Aは素子の最大電流を意味しない。
      | 未確認事項　　　　　; 実部品の温度上昇、SOA（電圧・電流・継続時間・温度で決まる安全動作範囲）、遮断時間、寄生要素を含む過渡動作。メーカーの用途説明と、現回路での成立確認は別に扱う。
      | 
      | 仕様・用途出典　　　; Infineon IPB048N15N5LFデータシート Rev.2.2（2022-09-09）、p.1（用途）、p.3～4（定格・特性）、p.6（SOA）。
      | https://www.infineon.com/assets/row/public/documents/24/49/infineon-ipb048n15n5lf-datasheet-en.pdf
      | 制御動作の出典　　　; Analog Devices LTC4364-1/LTC4364-2データシート Rev.B、p.8、p.11～12（端子機能・動作）。
      | https://www.analog.com/media/en/technical-documentation/data-sheets/ltc4364-1-4364-2.pdf
      | 
      | 今回の整理　　　　　; 部品番号・接続・メーカー仕様・近似条件を含む既存説明を保持。項目の区切り位置と表示名を整理する。
      | 
      | 【この説明欄の略語・記号】
      | 用語1　　　　　　　 ; IC：Integrated Circuit（集積回路）。複数の電子素子と機能を小さな半導体チップに集積した部品。
      | 用語2　　　　　　　 ; PWM：Pulse Width Modulation（パルス幅変調）。周期に対するON時間の割合を変えて、スイッチの平均的な電力伝達を調整する方式。
      | 用語3　　　　　　　 ; MOSFET：Metal-Oxide-Semiconductor Field-Effect Transistor（金属・酸化膜・半導体構造の電界効果トランジスタ）。ゲートとソースの電圧でドレインとソースの導通を制御する素子。N-MOSはNチャネル型を表す。
      | 用語4　　　　　　　 ; SOA：Safe Operating Area（安全動作領域）。素子が扱える電圧・電流・継続時間・温度の組合せ。耐圧や最大電流を個別に満たすだけではSOAの成立にならない。
      | 用語5　　　　　　　 ; VGS：Gate-to-Source Voltage（ゲート・ソース間電圧）。ゲートの電圧をソース基準で表す。GND基準のゲート電圧とは同じとは限らない。
      | 用語6　　　　　　　 ; VDS：Drain-to-Source Voltage（ドレイン・ソース間電圧）。MOSFETの主電流端子間にかかる電圧。
      | 用語7　　　　　　　 ; ID：Drain Current（ドレイン電流）。MOSFETのドレインを流れる電流。Idというモデル設定値は校正条件である場合があり、最大電流定格とは区別する。
      | 用語8　　　　　　　 ; Ciss：Input Capacitance（入力容量）。MOSFETの入力側の等価容量。測定条件に依存する。
      | 用語9　　　　　　　 ; Coss：Output Capacitance（出力容量）。MOSFETの出力側の等価容量。ドレイン・ソース電圧に依存する。
      | 用語10　　　　　　　; Crss：Reverse Transfer Capacitance（帰還容量）。主にゲート・ドレイン間の容量。スイッチング時の電圧変化がゲートへ結合する要因。
      | 用語11　　　　　　　; LeadRg：Gate lead resistance（モデル内のゲート側直列抵抗パラメータ）。このモデルで内部ゲート抵抗をまとめて与える設定名。パッケージのリード単独の抵抗という保証値ではない。
      | 用語12　　　　　　　; GND：Ground（回路の基準電位・電流帰路）。この図の共通基準。保護接地や大地への接続を意味するとは限らない。
      | 用語13　　　　　　　; SHDN：Shutdown（停止制御端子）。LTC4364ではLowで停止を指示する。Highは動作許可であり、保護判定を無効にするものではない。
      | 用語14　　　　　　　; OV：Overvoltage（過電圧検出）。LTC4364の入力側過電圧判定。FBで行う出力電圧制限とは機能が異なる。
      | 用語15　　　　　　　; FB：Feedback（帰還）。出力などを検出して内部制御へ戻すための信号・端子。
      | 用語16　　　　　　　; VIN/VOUT：入力電圧・出力電圧を表す端子／ネット名。INは入力、OUTは出力。電源変換器の電力端子なのか、検出用端子なのかは対象部品によって異なるため、端子と接続の説明に従う。
      | 用語17　　　　　　　; VCC/VDD/VEE/VS：ICの電源端子名。文字の歴史的な由来を現在の接続機能へ当てはめない。現回路のVEEはU8/U10では浮動基準SW、U9ではGND。各電圧・基準は端子と接続を参照する。
      | 用語18　　　　　　　; HGATE/DGATE：LTC4364の二つの外付けMOSFETゲート駆動出力。HGATEは主に電圧・電流制限側のP_Q1、DGATEは理想ダイオード／逆流防止側のP_Q2を駆動する。主電力段の上下PWMとは別の仕組み。
      | 用語19　　　　　　　; SW：Switching Node（スイッチング点）。主電力段の上下MOSFETとL1がつながる、電圧が高速に切り替わる点。GNDとは別電位。
  M2_FDB3632_APPROX : ee_lib/Semiconductors & Converters/N-Channel MOSFET  Description=|  paramTerminal=ee.enum.mosfet.numberOfTerminals.three  parameterization=ee.enum.mosfet.parameterization.datasheet  Beta=5.0 A/V^2  Rds=0.0048 Ohm  Id=4 A  Vgs=10 V  Vth=4.1 V  Vth0=1.7 V  lam=0 1/V  gamma_vth=0.5 V^(1/2)  phib=0.5 V  Vth1=1.9071 V  Vbs1=-1 V  Vth2=2.066 V  Vbs2=-2 V  Tmeas=25 degC  Vgs_vec=[-1, -.5, 2, 3, 4, 5] V  Vds_vec=[0, 2, 4, 8, 12, 16, 20] V  Vbs_vec=[0, -4, -6, -12] V  T_vec=[25, 125] degC  Vth_vec=[.4, 1.2, 1.4, 1.45] V  Vth_mat=[.4, .35; 1.2, 1.15; 1.4, 1.35; 1.45, 1.4] V  Ids_mat=[0, 0, 0, 0, 0, 0, 0; 0, 0, 0, 0, 0, 0, 0; 0, .003, .0038, .0043, .0046, .0048, .0049; 0, .0055, .008, .009, .0095, .01, .0101; 0, .0115, .016, .018, .019, .0195, .02; 0, .0152, .0225, .0265, .028, .0295, .03] A  Ids_mat0=[0, 0, 0, 0, 0, 0, 0; 0, 0, 0, 0, 0, 0, 0; 0, .003, .0038, .0043, .0046, .0048, .0049; 0, .0055, .008, .009, .0095, .01, .0101; 0, .0115, .016, .018, .019, .0195, .02; 0, .0152, .0225, .0265, .028, .0295, .03] A  Ids_mat_3D=zeros(6, 7, 2) A  Ids_mat_3D0=zeros(6, 7, 2) A  IV_table_symmetry=ee.enum.mosfet.symmetricNIV.no  RS=0.0001 Ohm  RD=0.0001 Ohm  RB=0.001 Ohm  LeadRs=0 Ohm  LeadRd=0 Ohm  LeadRg=25 Ohm  LeadRb=0 Ohm  LS=0 nH  LD=0 nH  LG=0 nH  LB=0 nH  C_param=ee.enum.mosfet.capacitanceParam.fixedciss  C_GS=270 pF  C_GD=80 pF  C_GB=0 pF  C_DS=0 pF  C_iss=290e-12 F  C_rss=13e-12 F  C_oss=1400e-12 F  C_iss_vec=[720, 700, 590, 470, 390, 310] pF  C_rss_vec=[450, 400, 300, 190, 95, 55] pF  C_oss_vec=[900, 810, 690, 420, 270, 170] pF  C_GS_vec=[270, 300, 290, 280, 295, 255] pF  C_GD_vec=[450, 400, 300, 190, 95, 55] pF  C_GB_vec=[270, 300, 290, 280, 295, 255] pF  C_Vgs_vec=0 V  C_DS_vec=[450, 410, 390, 230, 175, 115] pF  C_Vds_vec=[.1, .3, 1, 3, 10, 30] V  V_GS_for_cap_data=0 V  charge_linearity_param=ee.enum.mosfet.cgdLinearity.constant  C_OX=200 pF  V_C_OX=-0.5 V  charge_linearity_param_vgb=ee.enum.mosfet.cgbLinearity.instantly  charge_linearity_param_with_vgb=ee.enum.mosfet.cgbLinearityWithSeparateCgb.instantly  Di_param=ee.enum.mosfet.diodeParam.exponential  IsDiode=1e-9 A  Vbi=0.6 V  n=1.5  Cj0Diode=0 pF  TT=0 s  Tmeas_dio=25 degC  TableTypeNoT=ee.enum.mosfet.tableType.IfMat  TableType=ee.enum.diode.tableType.IfMat  IfVec=[.07, .12, .19, 1.75, 4.24, 7.32, 11.2] A  IfMat=[.07, .12, .19, 1.75, 4.24, 7.32, 11.2; .16, .3, .72, 2.14, 4.02, 6.35, 9.12] A  VfVecV=[.9, 1.15, 1.25, 1.5, 1.75, 2.17, 2.6, 2.85] V  VfMatV=[.9, 1.15, 1.25, 1.5, 1.75, 2.17, 2.6, 2.85; .58, .68, .75, 1.1, 1.38, 1.77, 2.27, 2.7] V  TjVec=[25, 125] degC  VfVec=[.5, .7, .9, 1.3, 1.7, 2.1, 2.5] V  IfVecV=[.1, .2, .5, 1, 2, 4, 7, 10] A  diode_Goff=1e-12 1/Ohm  prmDatasheet=ee.enum.temperatureParameterization.none  prmEquCoeff=ee.enum.temperatureParameterization.none  dVth_dT=-6 mV/K  dVth0_dT=-6 mV/K  Rds_T2=0.037 Ohm  BEXDatasheet=-1.5  BEXEquCoeff=-1.5  etaisDatasheet=3  etaisEquCoeff=3  Tmeas2=125 degC  etaisTabulated=3  TdeviceDatasheet=25 degC  TdeviceEquCoeff=25 degC  TdeviceTabulated=25 degC  i_g_specify=off  i_g_priority=None  i_g=0 A  i_g_nominal_specify=off  i_g_nominal_value=1  i_g_nominal_unit=A  i_d_specify=off  i_d_priority=None  i_d=0 A  i_d_nominal_specify=off  i_d_nominal_value=1  i_d_nominal_unit=A  i_b_specify=off  i_b_priority=None  i_b=0 A  i_b_nominal_specify=off  i_b_nominal_value=1  i_b_nominal_unit=A  voltage_gs_specify=off  voltage_gs_priority=None  voltage_gs=0 V  voltage_gs_nominal_specify=off  voltage_gs_nominal_value=1  voltage_gs_nominal_unit=V  voltage_ds_specify=off  voltage_ds_priority=None  voltage_ds=0 V  voltage_ds_nominal_specify=off  voltage_ds_nominal_value=1  voltage_ds_nominal_unit=V  voltage_bs_specify=off  voltage_bs_priority=None  voltage_bs=0 V  voltage_bs_nominal_specify=off  voltage_bs_nominal_value=1  voltage_bs_nominal_unit=V  v_Cgs_specify=off  v_Cgs_priority=High  v_Cgs=0 V  v_Cgs_nominal_specify=off  v_Cgs_nominal_value=1  v_Cgs_nominal_unit=V  v_Cds_specify=off  v_Cds_priority=High  v_Cds=0 V  v_Cds_nominal_specify=off  v_Cds_nominal_value=1  v_Cds_nominal_unit=V  v_Cbs_specify=off  v_Cbs_priority=High  v_Cbs=0 V  v_Cbs_nominal_specify=off  v_Cbs_nominal_value=1  v_Cbs_nominal_unit=V  thermal_network_parameterization=ee.enum.thermalNetworkTopology.junctionCase  Rth=[0, 10] K/W  Rth_Cauer=[1, 3, 10] K/W  Rth_Foster=[.08, .14, .22, .16] K/W  thermal_mass_parameterization=ee.enum.thermalNetwork.timeconstant  thermal_mass=[0, 1] J/K  thermal_mass_Cauer=[.1, .3, 1] J/K  thermal_mass_Foster=[.001, .005, .05, .5] J/K  thermal_time_constant=[0, 10] s  thermal_time_constant_Cauer=[1, 3, 10] s  thermal_time_constant_Foster=[7e-05, .0007, .01, .08] s  thermal_mass_initial_temperatures=[25, 25] degC  thermal_mass_initial_temperatures_Cauer=[25, 25, 25] degC  Tvec_initial_Foster=[25, 25, 25, 25] degC  betaref=18 A/V^2  Vfbref=-1.1 V  gamma=3.5 V^(1/2)  phib2ref=1 V  thesatref=0.4 1/V  alpha=0  Vp=5e-2 V  thesrref=0 1/V  m=8  Tref=25 degC  Rsref=2e-3 Ohm  Rdref=0.17 Ohm  Rgref=8.4 Ohm  Rbref=2e-3 Ohm  Cox=1500 pF  Cgso=100 pF  Cgdo=14 pF  Isref=5.2e-13 A  Cj0=480 pF  Tprm=ee.enum.temperatureParameterization.none  etabet=1.3  Stvfb=5e-4 V/K  Stphib=-8.5e-4 V/K  etasat=1.04  etasr=0.65  etar=0.95  etais=3  Tsim=25 degC  Ig_specify=off  Ig_priority=None  Ig=0 A  Ig_nominal_specify=off  Ig_nominal_value=1  Ig_nominal_unit=nA  Ids_specify=off  Ids_priority=None  Ids=0 A  Ids_nominal_specify=off  Ids_nominal_value=1  Ids_nominal_unit=A  Ib_specify=off  Ib_priority=None  Ib=0 A  Ib_nominal_specify=off  Ib_nominal_value=1  Ib_nominal_unit=uA  V_gs_specify=off  V_gs_priority=None  V_gs=0 V  V_gs_nominal_specify=off  V_gs_nominal_value=1  V_gs_nominal_unit=V  V_ds_specify=off  V_ds_priority=None  V_ds=0 V  V_ds_nominal_specify=off  V_ds_nominal_value=1  V_ds_nominal_unit=V  V_bs_specify=off  V_bs_priority=None  V_bs=0 V  V_bs_nominal_specify=off  V_bs_nominal_value=1  V_bs_nominal_unit=V  QGoverCox_specify=off  QGoverCox_priority=None  QGoverCox=0 V  QGoverCox_nominal_specify=off  QGoverCox_nominal_value=1  QGoverCox_nominal_unit=V  QDoverCox_specify=off  QDoverCox_priority=None  QDoverCox=0 V  QDoverCox_nominal_specify=off  QDoverCox_nominal_value=1  QDoverCox_nominal_unit=V  QBoverCox_specify=off  QBoverCox_priority=None  QBoverCox=0 V  QBoverCox_nominal_specify=off  QBoverCox_nominal_value=1  QBoverCox_nominal_unit=V  T0=[25, 25] degC  T0_Cauer=[25, 25, 25] degC
      | この回路での名前　　; P_Q2
      | 部品名　　　　　　　; IPB048N15N5LFATMA1
      | この回路での役割　　; 電池から充電器へ向かう逆流を止めるための保護用MOSFET。
      | ここでの動き　　　　; 通常の充電方向では低い抵抗で電流を通すよう保護IC P_U1が制御し、逆流する条件ではOFFへ向かわせる。P_Q1とソースを共通にして組み合わせる。
      | 
      | 【詳しい働き・仕様・接続・確認の範囲】
      | 部品種別　　　　　　; 逆流防止用NチャネルMOSFET
      | 公称値　　　　　　　; 150V / 4.8mOhm max at25C10V
      | 配置目的　　　　　　; P_Q1と共通ソースで組み合わせ、電池から充電器へ向かう逆流をLTC4364のDGATE制御で抑える。
      | 意図する動作　　　　; 通常の順方向通電では低いON抵抗を使い、逆向き電流が生じる条件ではゲートを下げる。ゲート制御はPWMではない。高速遮断時間・逆流ピークは現固定容量モデルだけでは実部品保証にならない。
      | 端子と接続　　　　　; G G → P_DGATE、D D → P_SENSE、S S → P_SOURCE
      | 
      | 制御担当　　　　　　; LTC4364のDGATE側。P_Q1を制御するHGATEとは別経路。
      | 共通ソース　　　　　; P_Q1とP_Q2のソースはP_SOURCEで共通。GNDとは異なる。
      | メーカー用途との関係; 同じ150 V linear-mode品を割り当てているが、P_Q2の主目的は逆流防止。品種の用途説明だけで高速遮断・逆流ピーク・SOAの適合を保証しない。
      | 
      | 部品種別　　　　　　; NチャネルMOSFET（逆流防止経路用）。
      | 部品分類　　　　　　; 150 V linear-mode MOSFET（リニア動作を考慮した品種）。
      | メーカー　　　　　　; Infineon。
      | 部品名の補足　　　　; IPB048N15N5LFATMA1（基本型番：IPB048N15N5LF）。
      | 採用状態　　　　　　; 現モデルへ割り当てた実部品候補。実部品としての全条件での成立確認は未完了。
      | 
      | 耐圧　　　　　　　　; ドレイン－ソース間150 V。端子間電圧の定格であり、この値だけで回路全体の安全性は判断しない。
      | 導通時抵抗　　　　　; 最大4.8 mΩ、代表3.9 mΩ。測定条件は接合温度25 ℃、ゲート－ソース電圧10 V、ドレイン電流100 A。
      | 内部ゲート抵抗　　　; 代表25 Ω、最大38 Ω。メーカーの設計規定値であり、出荷時の全数測定値ではない。
      | 総ゲート電荷　　　　; 代表84 nC。VDD=75 V、ID=60 A、VGS=0→10 Vの条件。
      | 
      | モデル抵抗近似　　　; 内部ゲート抵抗の代表値25 Ωを、SimscapeのGate lead resistance（LeadRg）にまとめて近似している。外付け抵抗を25 Ω追加した意味でも、パッケージのリードだけが25 Ωという意味でもない。
      | モデル容量近似　　　; VGS=0 V、VDS=75 V、1 MHzでの代表容量Ciss=290 pF、Coss=1400 pF、Crss=13 pFを固定値として使う。電圧で変化する容量や総ゲート電荷84 nCを再現したモデルではない。
      | モデル導通特性　　　; 現在のモデルの校正用電流パラメータIdは4 Aであり、ON抵抗のメーカー測定条件100 Aと一致していない。4 Aは素子の最大電流を意味しない。
      | 未確認事項　　　　　; 実部品の温度上昇、SOA（電圧・電流・継続時間・温度で決まる安全動作範囲）、遮断時間、寄生要素を含む過渡動作。メーカーの用途説明と、現回路での成立確認は別に扱う。
      | 
      | 仕様・用途出典　　　; Infineon IPB048N15N5LFデータシート Rev.2.2（2022-09-09）、p.1（用途）、p.3～4（定格・特性）、p.6（SOA）。
      | https://www.infineon.com/assets/row/public/documents/24/49/infineon-ipb048n15n5lf-datasheet-en.pdf
      | 制御動作の出典　　　; Analog Devices LTC4364-1/LTC4364-2データシート Rev.B、p.8、p.11～12（端子機能・動作）。
      | https://www.analog.com/media/en/technical-documentation/data-sheets/ltc4364-1-4364-2.pdf
      | 
      | 【この説明欄の略語・記号】
      | 用語1　　　　　　　 ; IC：Integrated Circuit（集積回路）。複数の電子素子と機能を小さな半導体チップに集積した部品。
      | 用語2　　　　　　　 ; PWM：Pulse Width Modulation（パルス幅変調）。周期に対するON時間の割合を変えて、スイッチの平均的な電力伝達を調整する方式。
      | 用語3　　　　　　　 ; MOSFET：Metal-Oxide-Semiconductor Field-Effect Transistor（金属・酸化膜・半導体構造の電界効果トランジスタ）。ゲートとソースの電圧でドレインとソースの導通を制御する素子。N-MOSはNチャネル型を表す。
      | 用語4　　　　　　　 ; SOA：Safe Operating Area（安全動作領域）。素子が扱える電圧・電流・継続時間・温度の組合せ。耐圧や最大電流を個別に満たすだけではSOAの成立にならない。
      | 用語5　　　　　　　 ; VGS：Gate-to-Source Voltage（ゲート・ソース間電圧）。ゲートの電圧をソース基準で表す。GND基準のゲート電圧とは同じとは限らない。
      | 用語6　　　　　　　 ; VDS：Drain-to-Source Voltage（ドレイン・ソース間電圧）。MOSFETの主電流端子間にかかる電圧。
      | 用語7　　　　　　　 ; ID：Drain Current（ドレイン電流）。MOSFETのドレインを流れる電流。Idというモデル設定値は校正条件である場合があり、最大電流定格とは区別する。
      | 用語8　　　　　　　 ; Ciss：Input Capacitance（入力容量）。MOSFETの入力側の等価容量。測定条件に依存する。
      | 用語9　　　　　　　 ; Coss：Output Capacitance（出力容量）。MOSFETの出力側の等価容量。ドレイン・ソース電圧に依存する。
      | 用語10　　　　　　　; Crss：Reverse Transfer Capacitance（帰還容量）。主にゲート・ドレイン間の容量。スイッチング時の電圧変化がゲートへ結合する要因。
      | 用語11　　　　　　　; LeadRg：Gate lead resistance（モデル内のゲート側直列抵抗パラメータ）。このモデルで内部ゲート抵抗をまとめて与える設定名。パッケージのリード単独の抵抗という保証値ではない。
      | 用語12　　　　　　　; GND：Ground（回路の基準電位・電流帰路）。この図の共通基準。保護接地や大地への接続を意味するとは限らない。
      | 用語13　　　　　　　; VCC/VDD/VEE/VS：ICの電源端子名。文字の歴史的な由来を現在の接続機能へ当てはめない。現回路のVEEはU8/U10では浮動基準SW、U9ではGND。各電圧・基準は端子と接続を参照する。
      | 用語14　　　　　　　; HGATE/DGATE：LTC4364の二つの外付けMOSFETゲート駆動出力。HGATEは主に電圧・電流制限側のP_Q1、DGATEは理想ダイオード／逆流防止側のP_Q2を駆動する。主電力段の上下PWMとは別の仕組み。
      | 用語15　　　　　　　; SW：Switching Node（スイッチング点）。主電力段の上下MOSFETとL1がつながる、電圧が高速に切り替わる点。GNDとは別電位。
  R1_205k : fl_lib/Electrical/Electrical Elements/Resistor  Description=|  R=243000 Ohm  i_specify=off  i_priority=None  i=0 A  i_nominal_specify=off  i_nominal_value=1  i_nominal_unit=A  v_specify=off  v_priority=None  v=0 V  v_nominal_specify=off  v_nominal_value=1  v_nominal_unit=V
      | この回路での名前　　; P_R1
      | 部品名　　　　　　　; TNPW0805243KBEEA
      | この回路での役割　　; 充電器から保護回路へ入る電圧が、起動してよい範囲にあるかを判断するための分圧抵抗。
      | ここでの動き　　　　; 保護IC LTC4364へ高い電圧をそのまま入れず、P_R2・P_R3と一緒に小さくした電圧を渡す。243 kΩの本品が分圧列の高電圧側を受け持つ。内部の古い名前に205kとあっても、現在値は243 kΩである。
      | 
      | 【詳しい働き・仕様・接続・確認の範囲】
      | 部品種別　　　　　　; 保護入力UV/OV分圧上側抵抗
      | 公称値　　　　　　　; 243 kΩ
      | 配置目的　　　　　　; VOUTからP_UVへ接続し、P_R2/P_R3とともに起動条件の入力電圧分圧を構成する。
      | 意図する動作　　　　; 部品値は243 kΩ。旧内部名205kは現在値ではない。
      | 端子と接続　　　　　; 1 1 → VOUT、2 2 → P_UV
      | 部品の耐圧　　　　　; 150 V（既存メーカー資料照合記録の定格。回路全体の適合とは別。）
      | 公称値の公差　　　　; ±0.1%（既存部品資料の値）
      | 部品資料の根拠　　　; Vishay TNPW e3データシート28758の抵抗値範囲・注文型番構成との照合記録。価格や在庫を確認した意味ではない。
      | モデルの範囲　　　　; Simscape抵抗の集中定数表現。部品の許容差、定格電力、温度係数、寄生インダクタンスの適合を示すものではない。
      | モデル設定　　　　　; R=243 kΩ。これらは保存モデルの設定値であり、すべてが実部品の保証値という意味ではない。
      | 確認の範囲　　　　　; 本説明は保存回路の部品情報・端子割当・既存設計意図を整理したもの。今回の説明更新によって新たな動作試験や実機検証を実施した意味ではない。
      | 設計記録　　　　　　; evaluation\component_annotations_20261022_r01\before_graph.json
      | evaluation\component_annotations_20261022_r01\before_metadata.json
      | evaluation\protection_capacitor_integration_20261021_r01\final_delivery\independent_readback\physical_bom.json
      | evaluation\protection_capacitor_integration_20261021_r01\protection_review\component_net_map.json
      | 
      | 【この説明欄の略語・記号】
      | 用語1　　　　　　　 ; UV：Undervoltage（低電圧検出）。LTC4364の入力電圧が低い状態を判定する端子。
      | 用語2　　　　　　　 ; OV：Overvoltage（過電圧検出）。LTC4364の入力側過電圧判定。FBで行う出力電圧制限とは機能が異なる。
      | 用語3　　　　　　　 ; FB：Feedback（帰還）。出力などを検出して内部制御へ戻すための信号・端子。
      | 用語4　　　　　　　 ; VIN/VOUT：入力電圧・出力電圧を表す端子／ネット名。INは入力、OUTは出力。電源変換器の電力端子なのか、検出用端子なのかは対象部品によって異なるため、端子と接続の説明に従う。
  R2_3k92 : fl_lib/Electrical/Electrical Elements/Resistor  Description=|  R=2740 Ohm  i_specify=off  i_priority=None  i=0 A  i_nominal_specify=off  i_nominal_value=1  i_nominal_unit=A  v_specify=off  v_priority=None  v=0 V  v_nominal_specify=off  v_nominal_value=1  v_nominal_unit=V
      | この回路での名前　　; P_R2
      | 部品名　　　　　　　; TNPW08052K74BEEA
      | この回路での役割　　; 保護IC LTC4364が「電圧が低すぎる」と「高すぎる」を、別々の条件で判断できるようにするための抵抗。
      | ここでの動き　　　　; P_R1・P_R3と並ぶ分圧列の途中に入り、二つの電圧検出点の間に差を作る。この差と抵抗全体の比によって判定範囲を設定する。実際のしきい値には抵抗とICの誤差も含まれる。
      | 
      | 【詳しい働き・仕様・接続・確認の範囲】
      | 部品種別　　　　　　; 保護入力UV/OV分圧中間抵抗
      | 公称値　　　　　　　; 2.74 kΩ
      | 配置目的　　　　　　; P_UV–P_OV間に入り、UVとOVの異なるしきい値を同じ分圧列から作る。
      | 意図する動作　　　　; 部品値は2.74 kΩ。抵抗比・比較器しきい値・ヒステリシスの誤差で実検出点が変わる。
      | 端子と接続　　　　　; 1 1 → P_UV、2 2 → P_OV
      | 部品の耐圧　　　　　; 150 V（既存メーカー資料照合記録の定格。回路全体の適合とは別。）
      | 公称値の公差　　　　; ±0.1%（既存部品資料の値）
      | 部品資料の根拠　　　; Vishay TNPW e3データシート28758の抵抗値範囲・注文型番構成との照合記録。価格や在庫を確認した意味ではない。
      | モデルの範囲　　　　; Simscape抵抗の集中定数表現。部品の許容差、定格電力、温度係数、寄生インダクタンスの適合を示すものではない。
      | モデル設定　　　　　; R=2.74 kΩ。これらは保存モデルの設定値であり、すべてが実部品の保証値という意味ではない。
      | 確認の範囲　　　　　; 本説明は保存回路の部品情報・端子割当・既存設計意図を整理したもの。今回の説明更新によって新たな動作試験や実機検証を実施した意味ではない。
      | 設計記録　　　　　　; evaluation\component_annotations_20261022_r01\before_graph.json
      | evaluation\component_annotations_20261022_r01\before_metadata.json
      | evaluation\protection_capacitor_integration_20261021_r01\final_delivery\independent_readback\physical_bom.json
      | evaluation\protection_capacitor_integration_20261021_r01\protection_review\component_net_map.json
      | 
      | 【この説明欄の略語・記号】
      | 用語1　　　　　　　 ; UV：Undervoltage（低電圧検出）。LTC4364の入力電圧が低い状態を判定する端子。
      | 用語2　　　　　　　 ; OV：Overvoltage（過電圧検出）。LTC4364の入力側過電圧判定。FBで行う出力電圧制限とは機能が異なる。
      | 用語3　　　　　　　 ; FB：Feedback（帰還）。出力などを検出して内部制御へ戻すための信号・端子。
  R3_3k48 : fl_lib/Electrical/Electrical Elements/Resistor  Description=|  R=4990 Ohm  i_specify=off  i_priority=None  i=0 A  i_nominal_specify=off  i_nominal_value=1  i_nominal_unit=A  v_specify=off  v_priority=None  v=0 V  v_nominal_specify=off  v_nominal_value=1  v_nominal_unit=V
      | この回路での名前　　; P_R3
      | 部品名　　　　　　　; TNPW08054K99BEEA
      | この回路での役割　　; 保護IC LTC4364へ渡す電圧検出信号を、共通GNDを基準として作るための抵抗。
      | ここでの動き　　　　; P_R1・P_R2と並ぶ分圧列の下側を4.99 kΩで共通GNDへつなぎ、入力電圧の判定比を決める。これは入力条件の判断用で、出力電圧を抑えるP_R7・P_R8の検出回路とは別の役割を持つ。
      | 
      | 【詳しい働き・仕様・接続・確認の範囲】
      | 部品種別　　　　　　; 保護入力UV/OV分圧下側抵抗
      | 公称値　　　　　　　; 4.99 kΩ
      | 配置目的　　　　　　; P_OVからGNDへ接続し、P_R1/P_R2とともに入力電圧判定比を定める。
      | 意図する動作　　　　; 部品値は4.99 kΩ。起動禁止判定とFBによる運転中の出力クランプを区別する。
      | 端子と接続　　　　　; 1 1 → P_OV、2 2 → GND
      | 部品の耐圧　　　　　; 150 V（既存メーカー資料照合記録の定格。回路全体の適合とは別。）
      | 公称値の公差　　　　; ±0.1%（既存部品資料の値）
      | 部品資料の根拠　　　; Vishay TNPW e3データシート28758の抵抗値範囲・注文型番構成との照合記録。価格や在庫を確認した意味ではない。
      | モデルの範囲　　　　; Simscape抵抗の集中定数表現。部品の許容差、定格電力、温度係数、寄生インダクタンスの適合を示すものではない。
      | モデル設定　　　　　; R=4.99 kΩ。これらは保存モデルの設定値であり、すべてが実部品の保証値という意味ではない。
      | 確認の範囲　　　　　; 本説明は保存回路の部品情報・端子割当・既存設計意図を整理したもの。今回の説明更新によって新たな動作試験や実機検証を実施した意味ではない。
      | 設計記録　　　　　　; evaluation\component_annotations_20261022_r01\before_graph.json
      | evaluation\component_annotations_20261022_r01\before_metadata.json
      | evaluation\protection_capacitor_integration_20261021_r01\final_delivery\independent_readback\physical_bom.json
      | evaluation\protection_capacitor_integration_20261021_r01\protection_review\component_net_map.json
      | 
      | 【この説明欄の略語・記号】
      | 用語1　　　　　　　 ; GND：Ground（回路の基準電位・電流帰路）。この図の共通基準。保護接地や大地への接続を意味するとは限らない。
      | 用語2　　　　　　　 ; UV：Undervoltage（低電圧検出）。LTC4364の入力電圧が低い状態を判定する端子。
      | 用語3　　　　　　　 ; OV：Overvoltage（過電圧検出）。LTC4364の入力側過電圧判定。FBで行う出力電圧制限とは機能が異なる。
      | 用語4　　　　　　　 ; FB：Feedback（帰還）。出力などを検出して内部制御へ戻すための信号・端子。
  R4_2k2 : fl_lib/Electrical/Electrical Elements/Resistor  Description=|  R=6800 Ohm  i_specify=off  i_priority=None  i=0 A  i_nominal_specify=off  i_nominal_value=1  i_nominal_unit=A  v_specify=off  v_priority=None  v=0 V  v_nominal_specify=off  v_nominal_value=1  v_nominal_unit=V
      | この回路での名前　　; P_R4
      | 部品名　　　　　　　; CRCW25126K80FKEG
      | この回路での役割　　; 保護IC LTC4364へ給電しつつ、その電源を制限するツェナーダイオードP_D1へ電流が流れすぎないようにするための抵抗。
      | ここでの動き　　　　; 充電器の出力から保護ICの電源へ入る経路に6.8 kΩを置き、電流を抑えながら電圧を落とす。抵抗での電圧降下が大きすぎるとICの動作電圧が足りなくなるため、電力損失と給電余裕を合わせて確認する。現在値は既存の候補設定。
      | 
      | 【詳しい働き・仕様・接続・確認の範囲】
      | 部品種別　　　　　　; 保護IC電源直列抵抗
      | 公称値　　　　　　　; 6.8 kΩ
      | 配置目的　　　　　　; VOUTからP_VCCへ給電し、P_D1のツェナー電流と故障時の持続消費電力を抑える。
      | 意図する動作　　　　; 6.8 kΩの候補。電圧降下はIC電源とタイマの動作にも影響するため、単に大きくすればよい部品ではない。熱・電源余裕の確認が残る。
      | 端子と接続　　　　　; 1 1 → VOUT、2 2 → P_VCC
      | 部品の耐圧　　　　　; 500 V（既存メーカー資料照合記録の定格。回路全体の適合とは別。）
      | 公称値の公差　　　　; ±1%（既存部品資料の値）
      | 部品資料の根拠　　　; Vishay D/CRCW e3データシート20035の抵抗値・注文型番構成との既存照合記録。実装後の熱・電圧適合とは別。
      | モデルの範囲　　　　; Simscape抵抗の集中定数表現。部品の許容差、定格電力、温度係数、寄生インダクタンスの適合を示すものではない。
      | モデル設定　　　　　; R=6.8 kΩ。これらは保存モデルの設定値であり、すべてが実部品の保証値という意味ではない。
      | 確認の範囲　　　　　; 本説明は保存回路の部品情報・端子割当・既存設計意図を整理したもの。今回の説明更新によって新たな動作試験や実機検証を実施した意味ではない。
      | 設計記録　　　　　　; evaluation\component_annotations_20261022_r01\before_graph.json
      | evaluation\component_annotations_20261022_r01\before_metadata.json
      | evaluation\protection_capacitor_integration_20261021_r01\final_delivery\independent_readback\physical_bom.json
      | evaluation\protection_capacitor_integration_20261021_r01\protection_review\component_net_map.json
      | 
      | 【この説明欄の略語・記号】
      | 用語1　　　　　　　 ; IC：Integrated Circuit（集積回路）。複数の電子素子と機能を小さな半導体チップに集積した部品。
      | 用語2　　　　　　　 ; MOSFET：Metal-Oxide-Semiconductor Field-Effect Transistor（金属・酸化膜・半導体構造の電界効果トランジスタ）。ゲートとソースの電圧でドレインとソースの導通を制御する素子。N-MOSはNチャネル型を表す。
      | 用語3　　　　　　　 ; GND：Ground（回路の基準電位・電流帰路）。この図の共通基準。保護接地や大地への接続を意味するとは限らない。
      | 用語4　　　　　　　 ; VIN/VOUT：入力電圧・出力電圧を表す端子／ネット名。INは入力、OUTは出力。電源変換器の電力端子なのか、検出用端子なのかは対象部品によって異なるため、端子と接続の説明に従う。
      | 用語5　　　　　　　 ; VCC/VDD/VEE/VS：ICの電源端子名。文字の歴史的な由来を現在の接続機能へ当てはめない。現回路のVEEはU8/U10では浮動基準SW、U9ではGND。各電圧・基準は端子と接続を参照する。
      | 用語6　　　　　　　 ; SW：Switching Node（スイッチング点）。主電力段の上下MOSFETとL1がつながる、電圧が高速に切り替わる点。GNDとは別電位。
  R5_10ohm : fl_lib/Electrical/Electrical Elements/Resistor  Description=|  R=10 Ohm  i_specify=off  i_priority=None  i=0 A  i_nominal_specify=off  i_nominal_value=1  i_nominal_unit=A  v_specify=off  v_priority=None  v=0 V  v_nominal_specify=off  v_nominal_value=1  v_nominal_unit=V
      | この回路での名前　　; P_R5
      | 部品名　　　　　　　; CRCW080510R0FKEA
      | この回路での役割　　; 保護用MOSFET P_Q1のゲートに出入りする電流を調整し、局所的な電圧の振動を抑えるための抵抗。
      | ここでの動き　　　　; 保護IC LTC4364とP_Q1のゲートの間に、外付けの10 Ωを入れる。ゲートの電荷が増減する速さに影響するため、遮断の速さや波形は別に確認する。MOSFET内部のゲート抵抗を表すモデル値とは区別する。
      | 
      | 【詳しい働き・仕様・接続・確認の範囲】
      | 部品種別　　　　　　; 保護直列MOSFETゲート抵抗
      | 公称値　　　　　　　; 10 Ω
      | 配置目的　　　　　　; LTC4364のHGATEとP_Q1ゲートの間に置き、局所的なゲート充放電・振動を調整する。
      | 意図する動作　　　　; 外付け10 Ωであり、P_Q1モデルへ近似した内部ゲート抵抗25 Ωとは別。
      | 端子と接続　　　　　; 1 1 → P_HGATE、2 2 → P_Q1_GATE
      | 公称値の公差　　　　; ±1%（既存部品資料の値）
      | 部品資料の根拠　　　; Vishay D/CRCW e3データシート20035の抵抗値・注文型番構成との既存照合記録。実装後の熱・電圧適合とは別。
      | モデルの範囲　　　　; Simscape抵抗の集中定数表現。部品の許容差、定格電力、温度係数、寄生インダクタンスの適合を示すものではない。
      | モデル設定　　　　　; R=10 Ω。これらは保存モデルの設定値であり、すべてが実部品の保証値という意味ではない。
      | 確認の範囲　　　　　; 本説明は保存回路の部品情報・端子割当・既存設計意図を整理したもの。今回の説明更新によって新たな動作試験や実機検証を実施した意味ではない。
      | 設計記録　　　　　　; evaluation\component_annotations_20261022_r01\before_graph.json
      | evaluation\component_annotations_20261022_r01\before_metadata.json
      | evaluation\protection_capacitor_integration_20261021_r01\final_delivery\independent_readback\physical_bom.json
      | evaluation\protection_capacitor_integration_20261021_r01\protection_review\component_net_map.json
      | 
      | 【この説明欄の略語・記号】
      | 用語1　　　　　　　 ; PWM：Pulse Width Modulation（パルス幅変調）。周期に対するON時間の割合を変えて、スイッチの平均的な電力伝達を調整する方式。
      | 用語2　　　　　　　 ; MOSFET：Metal-Oxide-Semiconductor Field-Effect Transistor（金属・酸化膜・半導体構造の電界効果トランジスタ）。ゲートとソースの電圧でドレインとソースの導通を制御する素子。N-MOSはNチャネル型を表す。
      | 用語3　　　　　　　 ; HGATE/DGATE：LTC4364の二つの外付けMOSFETゲート駆動出力。HGATEは主に電圧・電流制限側のP_Q1、DGATEは理想ダイオード／逆流防止側のP_Q2を駆動する。主電力段の上下PWMとは別の仕組み。
  R7_226k : fl_lib/Electrical/Electrical Elements/Resistor  Description=|  R=236000 Ohm  i_specify=off  i_priority=None  i=0 A  i_nominal_specify=off  i_nominal_value=1  i_nominal_unit=A  v_specify=off  v_priority=None  v=0 V  v_nominal_specify=off  v_nominal_value=1  v_nominal_unit=V
      | この回路での名前　　; P_R7
      | 部品名　　　　　　　; TNPW0805236KBEEA
      | この回路での役割　　; 保護回路が蓄電池側へ渡す電圧を上げすぎないよう、出力電圧を監視するための抵抗。
      | ここでの動き　　　　; 蓄電池側の電圧をP_R8と一緒に小さくして保護IC LTC4364へ返す。この帰還信号を使ってICが出力電圧を抑える設定を作る。236 kΩの本品が高電圧側を受け持つ。
      | 
      | 【詳しい働き・仕様・接続・確認の範囲】
      | 部品種別　　　　　　; 保護出力クランプ帰還上側抵抗
      | 公称値　　　　　　　; 236 kΩ
      | 配置目的　　　　　　; BAT_PLUSからP_FBへ接続し、P_R8とともに出力電圧クランプの帰還比を作る。
      | 意図する動作　　　　; 236 kΩ。入力側UV/OV判定とは独立した出力側の帰還。
      | 端子と接続　　　　　; 1 1 → BAT_PLUS、2 2 → P_FB
      | 部品の耐圧　　　　　; 150 V（既存メーカー資料照合記録の定格。回路全体の適合とは別。）
      | 公称値の公差　　　　; ±0.1%（既存部品資料の値）
      | 部品資料の根拠　　　; Vishay TNPW e3データシート28758の抵抗値範囲・注文型番構成との照合記録。価格や在庫を確認した意味ではない。
      | モデルの範囲　　　　; Simscape抵抗の集中定数表現。部品の許容差、定格電力、温度係数、寄生インダクタンスの適合を示すものではない。
      | モデル設定　　　　　; R=236 kΩ。これらは保存モデルの設定値であり、すべてが実部品の保証値という意味ではない。
      | 確認の範囲　　　　　; 本説明は保存回路の部品情報・端子割当・既存設計意図を整理したもの。今回の説明更新によって新たな動作試験や実機検証を実施した意味ではない。
      | 設計記録　　　　　　; evaluation\component_annotations_20261022_r01\before_graph.json
      | evaluation\component_annotations_20261022_r01\before_metadata.json
      | evaluation\protection_capacitor_integration_20261021_r01\final_delivery\independent_readback\physical_bom.json
      | evaluation\protection_capacitor_integration_20261021_r01\protection_review\component_net_map.json
      | 
      | 【この説明欄の略語・記号】
      | 用語1　　　　　　　 ; UV：Undervoltage（低電圧検出）。LTC4364の入力電圧が低い状態を判定する端子。
      | 用語2　　　　　　　 ; OV：Overvoltage（過電圧検出）。LTC4364の入力側過電圧判定。FBで行う出力電圧制限とは機能が異なる。
      | 用語3　　　　　　　 ; FB：Feedback（帰還）。出力などを検出して内部制御へ戻すための信号・端子。
  R8_4k02 : fl_lib/Electrical/Electrical Elements/Resistor  Description=|  R=4990 Ohm  i_specify=off  i_priority=None  i=0 A  i_nominal_specify=off  i_nominal_value=1  i_nominal_unit=A  v_specify=off  v_priority=None  v=0 V  v_nominal_specify=off  v_nominal_value=1  v_nominal_unit=V
      | この回路での名前　　; P_R8
      | 部品名　　　　　　　; TNPW08054K99BEEA
      | この回路での役割　　; 保護回路が出力電圧をどの高さで抑えるかを、P_R7と一緒に決めるための抵抗。
      | ここでの動き　　　　; 保護ICへ返す電圧検出点を4.99 kΩで共通GNDへつなぐ。P_R7との抵抗比とIC内部の基準値によって、出力電圧を抑え始める設定が決まる。実際のしきい値には双方の誤差が含まれる。
      | 
      | 【詳しい働き・仕様・接続・確認の範囲】
      | 部品種別　　　　　　; 保護出力クランプ帰還下側抵抗
      | 公称値　　　　　　　; 4.99 kΩ
      | 配置目的　　　　　　; P_FBからGNDへ接続し、P_R7とともにクランプ電圧設定を構成する。
      | 意図する動作　　　　; 4.99 kΩ。実しきい値には抵抗比とLTC4364基準値の誤差が入る。
      | 端子と接続　　　　　; 1 1 → P_FB、2 2 → GND
      | 部品の耐圧　　　　　; 150 V（既存メーカー資料照合記録の定格。回路全体の適合とは別。）
      | 公称値の公差　　　　; ±0.1%（既存部品資料の値）
      | 部品資料の根拠　　　; Vishay TNPW e3データシート28758の抵抗値範囲・注文型番構成との照合記録。価格や在庫を確認した意味ではない。
      | モデルの範囲　　　　; Simscape抵抗の集中定数表現。部品の許容差、定格電力、温度係数、寄生インダクタンスの適合を示すものではない。
      | モデル設定　　　　　; R=4.99 kΩ。これらは保存モデルの設定値であり、すべてが実部品の保証値という意味ではない。
      | 確認の範囲　　　　　; 本説明は保存回路の部品情報・端子割当・既存設計意図を整理したもの。今回の説明更新によって新たな動作試験や実機検証を実施した意味ではない。
      | 設計記録　　　　　　; evaluation\component_annotations_20261022_r01\before_graph.json
      | evaluation\component_annotations_20261022_r01\before_metadata.json
      | evaluation\protection_capacitor_integration_20261021_r01\final_delivery\independent_readback\physical_bom.json
      | evaluation\protection_capacitor_integration_20261021_r01\protection_review\component_net_map.json
      | 
      | 【この説明欄の略語・記号】
      | 用語1　　　　　　　 ; GND：Ground（回路の基準電位・電流帰路）。この図の共通基準。保護接地や大地への接続を意味するとは限らない。
      | 用語2　　　　　　　 ; FB：Feedback（帰還）。出力などを検出して内部制御へ戻すための信号・端子。
  RETURN_label_1 : ConnectionLabel  Description=|  Label=PROT_RETURN
      | この回路での名前　　; PROT_RETURN
      | 種別　　　　　　　　; ConnectionLabel
      | この回路での役割　　; 保護回路の帰路を、外側の共通GNDへ結ぶ。このラベルはプロトタイプという意味ではなく保護回路の戻り線を示す。明示的な境界端子を経由してBT1負極・PV1負極と同じノードになる。
      | 共通帰路の代表接続　; P_U1（保護MOSFETを制御する保護IC／LTC4364IMS-1#PBF）: GND
      |                     ; BT1（充電先の蓄電池／51.2V 100Ah LiFePO4）: -
      |                     ; PV1（直列太陽電池列の負極側パネル／400W panel 1/2）: -
      |                     ; U7（RP2040搭載Pico W／SC0918）: 3(GND), 8(GND), 13(GND), 18(GND), 23(GND), 28(GND), 33(AGND), 38(GND)
      |                     ; U1（外付けADC／MCP3208-CI/SL）: 8(CH7), 9(DGND), 14(AGND)
      | この場所の直接接続　; P_U1（保護MOSFETを制御する保護IC／LTC4364IMS-1#PBF）: GND
      | 直接接続の範囲　　　; このラベルから実際の線・分岐・明示的な境界端子だけを追った接続。同名ラベルによる離れた場所への接続はこの欄に含めない。
      | 同一ネット全端子　　; BT1: -
      |                     ; C1: 2(n)
      |                     ; C2: 2(n)
      |                     ; C3: 2(n)
      |                     ; C4: 2(n)
      |                     ; C7: 2(n)
      |                     ; C8: 2(n)
      |                     ; C9: 2(n)
      |                     ; C10: 2(n)
      |                     ; C13: 2(n)
      |                     ; C14: 2(n)
      |                     ; C15: 2(n)
      |                     ; C16: 2(n)
      |                     ; C17: 2
      |                     ; C18: 2
      |                     ; C19: 2
      |                     ; C20: 2
      |                     ; C21: 2
      |                     ; C22: 2
      |                     ; C23: 2
      |                     ; C24: 2
      |                     ; C25: 2
      |                     ; C26: 2
      |                     ; C27: 2
      |                     ; C28: 2
      |                     ; C29: 2
      |                     ; C30: 2
      |                     ; C31: 2
      |                     ; C33: 2
      |                     ; C34: 2
      |                     ; C35: 2
      |                     ; C36: 2
      |                     ; C40: 2
      |                     ; C41: 2
      |                     ; C42: 2
      |                     ; C43: 2
      |                     ; C44: 2
      |                     ; C45: 2
      |                     ; C46: 2
      |                     ; C47: 2
      |                     ; C48: 2
      |                     ; D2: 2(A)
      |                     ; PV1: -
      |                     ; P_CHG: N
      |                     ; P_COUT: N
      |                     ; P_CTMR: N
      |                     ; P_D1: A
      |                     ; P_R3: 2
      |                     ; P_R8: 2
      |                     ; P_RSHDN_PD: 2
      |                     ; P_U1: GND
      |                     ; Q2: 3(S)
      |                     ; Q3: 1(S1), 4(S2)
      |                     ; R1: 2(n)
      |                     ; R18: 2
      |                     ; R21: 2
      |                     ; R24: 2
      |                     ; R35: 2
      |                     ; R42: 2
      |                     ; R44: 2
      |                     ; R48: 2
      |                     ; U1: 8(CH7), 9(DGND), 14(AGND)
      |                     ; U2: 2(GND), 3(REF2), 4(RESERVED_GND)
      |                     ; U3: 2(GND), 3(REF2), 4(RESERVED_GND)
      |                     ; U4: 3(GND)
      |                     ; U5: 3(GND)
      |                     ; U6: 3(GND)
      |                     ; U7: 3(GND), 8(GND), 13(GND), 18(GND), 23(GND), 28(GND), 33(AGND), 38(GND)
      |                     ; U9: 4(VEE)
      |                     ; U10: 1(GNDP), 2(GNDP), 5(GNDP), 8(GNDP), 9(GNDP), 10(GNDP), 11(GNDP), 12(GNDP), 13(GNDP), 14(GNDP), 15(GNDP), 16(GNDP), 17(GNDP), 18(GNDP)
      |                     ; U11: 2(GND)
      |                     ; U12: 2(GND)
      | 接続部品数　　　　　; 72部品（部品番号で集計。同一ネット全体）
      | 接続端子数　　　　　; 99端子（423端子の部品対応表で集計。ラベル・境界ポートの重複は含めない）
      | この場所の端子数　　; 1端子／1部品（同名ラベルによる接続を除く）
      | 同階層同名ラベル数　; 8個（このラベル自身を含む）
      | 全階層の接続ラベル　; 87個（実際に同じノードへつながるラベル。名前が違う別名も含む）
      | 接続ルール　　　　　; 同じ階層の同じラベル名を仮想配線として結ぶ。別のSubsystem内とは名前だけでつながらず、明示的なConnection Portと配線をたどる。色は用途の表示であり接続を決めない。
      | 確認の範囲　　　　　; 現在の保存回路の端子・配線から求めた静的接続。抵抗やICの内部を導線として短絡せずに集計した。説明の更新は動作シミュレーション、タイミング、実部品の性能・実機動作を保証するものではない。
      | 記録の基準　　　　　; measurement_label_layout_20261022_r01/after_layout_graph.json。部品対応表は端子名の対応付けにのみ使用。
      | 
      | 【この説明欄の略語・記号】
      | 用語1　　　　　　　 ; ADC：Analog-to-Digital Converter（アナログ・デジタル変換器）。測定電圧をデジタル値へ変換する回路。電流や温度も、センサーで電圧へ変換した後に読み取る。
      | 用語2　　　　　　　 ; IC：Integrated Circuit（集積回路）。複数の電子素子と機能を小さな半導体チップに集積した部品。
      | 用語3　　　　　　　 ; CH：Channel（測定チャネル）。CH0〜CH7はADCの入力番号であり、同時測定を意味しない。
      | 用語4　　　　　　　 ; MOSFET：Metal-Oxide-Semiconductor Field-Effect Transistor（金属・酸化膜・半導体構造の電界効果トランジスタ）。ゲートとソースの電圧でドレインとソースの導通を制御する素子。N-MOSはNチャネル型を表す。
      | 用語5　　　　　　　 ; LiFePO4：Lithium Iron Phosphate（リン酸鉄リチウム）。電池の正極材料を示す化学式。英語の頭文字を並べた略語ではない。
      | 用語6　　　　　　　 ; GND：Ground（回路の基準電位・電流帰路）。この図の共通基準。保護接地や大地への接続を意味するとは限らない。
      | 用語7　　　　　　　 ; AGND：Analog Ground（アナログ回路の基準端子）。アナログ部分の電流帰路。現図では共通GNDへ接続されるが、実装時の電流経路への配慮は別途必要。
      | 用語8　　　　　　　 ; DGND：Digital Ground（デジタル回路の基準端子）。デジタル部分の電流帰路。現図では共通GNDへ接続される。
      | 用語9　　　　　　　 ; VREF/REF：基準電圧を表す端子名。REFはReference（基準）の意味。ADCの変換尺度や電流アンプの出力基準に使う。REF1/REF2の接続電位は個別に確認する。
      | 用語10　　　　　　　; VCC/VDD/VEE/VS：ICの電源端子名。文字の歴史的な由来を現在の接続機能へ当てはめない。現回路のVEEはU8/U10では浮動基準SW、U9ではGND。各電圧・基準は端子と接続を参照する。
      | 用語11　　　　　　　; GNDP：U10の一次側電源の基準端子。絶縁電源の入力側GND。二次側基準VEE=SWと直接同一の導体ではない。
      | 用語12　　　　　　　; SW：Switching Node（スイッチング点）。主電力段の上下MOSFETとL1がつながる、電圧が高速に切り替わる点。GNDとは別電位。
      | 用語13　　　　　　　; PROT_RETURN：保護回路の共通帰路。PROTはProtection（保護）、RETURNは帰路。プロトタイプの略ではなく、現回路では共通GNDへつながる。
  RETURN_label_2 : ConnectionLabel  Description=|  Label=PROT_RETURN
      | この回路での名前　　; PROT_RETURN
      | 種別　　　　　　　　; ConnectionLabel
      | この回路での役割　　; 保護回路の帰路を、外側の共通GNDへ結ぶ。このラベルはプロトタイプという意味ではなく保護回路の戻り線を示す。明示的な境界端子を経由してBT1負極・PV1負極と同じノードになる。
      | 共通帰路の代表接続　; P_U1（保護MOSFETを制御する保護IC／LTC4364IMS-1#PBF）: GND
      |                     ; BT1（充電先の蓄電池／51.2V 100Ah LiFePO4）: -
      |                     ; PV1（直列太陽電池列の負極側パネル／400W panel 1/2）: -
      |                     ; U7（RP2040搭載Pico W／SC0918）: 3(GND), 8(GND), 13(GND), 18(GND), 23(GND), 28(GND), 33(AGND), 38(GND)
      |                     ; U1（外付けADC／MCP3208-CI/SL）: 8(CH7), 9(DGND), 14(AGND)
      | この場所の直接接続　; P_R3（P_OVからGNDへ接続し、P_R1/P_R2とともに入力電圧判定比を定める／4.99 kΩ）: 2
      | 直接接続の範囲　　　; このラベルから実際の線・分岐・明示的な境界端子だけを追った接続。同名ラベルによる離れた場所への接続はこの欄に含めない。
      | 同一ネット全端子　　; BT1: -
      |                     ; C1: 2(n)
      |                     ; C2: 2(n)
      |                     ; C3: 2(n)
      |                     ; C4: 2(n)
      |                     ; C7: 2(n)
      |                     ; C8: 2(n)
      |                     ; C9: 2(n)
      |                     ; C10: 2(n)
      |                     ; C13: 2(n)
      |                     ; C14: 2(n)
      |                     ; C15: 2(n)
      |                     ; C16: 2(n)
      |                     ; C17: 2
      |                     ; C18: 2
      |                     ; C19: 2
      |                     ; C20: 2
      |                     ; C21: 2
      |                     ; C22: 2
      |                     ; C23: 2
      |                     ; C24: 2
      |                     ; C25: 2
      |                     ; C26: 2
      |                     ; C27: 2
      |                     ; C28: 2
      |                     ; C29: 2
      |                     ; C30: 2
      |                     ; C31: 2
      |                     ; C33: 2
      |                     ; C34: 2
      |                     ; C35: 2
      |                     ; C36: 2
      |                     ; C40: 2
      |                     ; C41: 2
      |                     ; C42: 2
      |                     ; C43: 2
      |                     ; C44: 2
      |                     ; C45: 2
      |                     ; C46: 2
      |                     ; C47: 2
      |                     ; C48: 2
      |                     ; D2: 2(A)
      |                     ; PV1: -
      |                     ; P_CHG: N
      |                     ; P_COUT: N
      |                     ; P_CTMR: N
      |                     ; P_D1: A
      |                     ; P_R3: 2
      |                     ; P_R8: 2
      |                     ; P_RSHDN_PD: 2
      |                     ; P_U1: GND
      |                     ; Q2: 3(S)
      |                     ; Q3: 1(S1), 4(S2)
      |                     ; R1: 2(n)
      |                     ; R18: 2
      |                     ; R21: 2
      |                     ; R24: 2
      |                     ; R35: 2
      |                     ; R42: 2
      |                     ; R44: 2
      |                     ; R48: 2
      |                     ; U1: 8(CH7), 9(DGND), 14(AGND)
      |                     ; U2: 2(GND), 3(REF2), 4(RESERVED_GND)
      |                     ; U3: 2(GND), 3(REF2), 4(RESERVED_GND)
      |                     ; U4: 3(GND)
      |                     ; U5: 3(GND)
      |                     ; U6: 3(GND)
      |                     ; U7: 3(GND), 8(GND), 13(GND), 18(GND), 23(GND), 28(GND), 33(AGND), 38(GND)
      |                     ; U9: 4(VEE)
      |                     ; U10: 1(GNDP), 2(GNDP), 5(GNDP), 8(GNDP), 9(GNDP), 10(GNDP), 11(GNDP), 12(GNDP), 13(GNDP), 14(GNDP), 15(GNDP), 16(GNDP), 17(GNDP), 18(GNDP)
      |                     ; U11: 2(GND)
      |                     ; U12: 2(GND)
      | 接続部品数　　　　　; 72部品（部品番号で集計。同一ネット全体）
      | 接続端子数　　　　　; 99端子（423端子の部品対応表で集計。ラベル・境界ポートの重複は含めない）
      | この場所の端子数　　; 1端子／1部品（同名ラベルによる接続を除く）
      | 同階層同名ラベル数　; 8個（このラベル自身を含む）
      | 全階層の接続ラベル　; 87個（実際に同じノードへつながるラベル。名前が違う別名も含む）
      | 接続ルール　　　　　; 同じ階層の同じラベル名を仮想配線として結ぶ。別のSubsystem内とは名前だけでつながらず、明示的なConnection Portと配線をたどる。色は用途の表示であり接続を決めない。
      | 確認の範囲　　　　　; 現在の保存回路の端子・配線から求めた静的接続。抵抗やICの内部を導線として短絡せずに集計した。説明の更新は動作シミュレーション、タイミング、実部品の性能・実機動作を保証するものではない。
      | 記録の基準　　　　　; measurement_label_layout_20261022_r01/after_layout_graph.json。部品対応表は端子名の対応付けにのみ使用。
      | 
      | 【この説明欄の略語・記号】
      | 用語1　　　　　　　 ; ADC：Analog-to-Digital Converter（アナログ・デジタル変換器）。測定電圧をデジタル値へ変換する回路。電流や温度も、センサーで電圧へ変換した後に読み取る。
      | 用語2　　　　　　　 ; IC：Integrated Circuit（集積回路）。複数の電子素子と機能を小さな半導体チップに集積した部品。
      | 用語3　　　　　　　 ; CH：Channel（測定チャネル）。CH0〜CH7はADCの入力番号であり、同時測定を意味しない。
      | 用語4　　　　　　　 ; MOSFET：Metal-Oxide-Semiconductor Field-Effect Transistor（金属・酸化膜・半導体構造の電界効果トランジスタ）。ゲートとソースの電圧でドレインとソースの導通を制御する素子。N-MOSはNチャネル型を表す。
      | 用語5　　　　　　　 ; LiFePO4：Lithium Iron Phosphate（リン酸鉄リチウム）。電池の正極材料を示す化学式。英語の頭文字を並べた略語ではない。
      | 用語6　　　　　　　 ; GND：Ground（回路の基準電位・電流帰路）。この図の共通基準。保護接地や大地への接続を意味するとは限らない。
      | 用語7　　　　　　　 ; AGND：Analog Ground（アナログ回路の基準端子）。アナログ部分の電流帰路。現図では共通GNDへ接続されるが、実装時の電流経路への配慮は別途必要。
      | 用語8　　　　　　　 ; DGND：Digital Ground（デジタル回路の基準端子）。デジタル部分の電流帰路。現図では共通GNDへ接続される。
      | 用語9　　　　　　　 ; OV：Overvoltage（過電圧検出）。LTC4364の入力側過電圧判定。FBで行う出力電圧制限とは機能が異なる。
      | 用語10　　　　　　　; FB：Feedback（帰還）。出力などを検出して内部制御へ戻すための信号・端子。
      | 用語11　　　　　　　; VREF/REF：基準電圧を表す端子名。REFはReference（基準）の意味。ADCの変換尺度や電流アンプの出力基準に使う。REF1/REF2の接続電位は個別に確認する。
      | 用語12　　　　　　　; VCC/VDD/VEE/VS：ICの電源端子名。文字の歴史的な由来を現在の接続機能へ当てはめない。現回路のVEEはU8/U10では浮動基準SW、U9ではGND。各電圧・基準は端子と接続を参照する。
      | 用語13　　　　　　　; GNDP：U10の一次側電源の基準端子。絶縁電源の入力側GND。二次側基準VEE=SWと直接同一の導体ではない。
      | 用語14　　　　　　　; SW：Switching Node（スイッチング点）。主電力段の上下MOSFETとL1がつながる、電圧が高速に切り替わる点。GNDとは別電位。
      | 用語15　　　　　　　; PROT_RETURN：保護回路の共通帰路。PROTはProtection（保護）、RETURNは帰路。プロトタイプの略ではなく、現回路では共通GNDへつながる。
  RETURN_label_3 : ConnectionLabel  Description=|  Label=PROT_RETURN
      | この回路での名前　　; PROT_RETURN
      | 種別　　　　　　　　; ConnectionLabel
      | この回路での役割　　; 保護回路の帰路を、外側の共通GNDへ結ぶ。このラベルはプロトタイプという意味ではなく保護回路の戻り線を示す。明示的な境界端子を経由してBT1負極・PV1負極と同じノードになる。
      | 共通帰路の代表接続　; P_U1（保護MOSFETを制御する保護IC／LTC4364IMS-1#PBF）: GND
      |                     ; BT1（充電先の蓄電池／51.2V 100Ah LiFePO4）: -
      |                     ; PV1（直列太陽電池列の負極側パネル／400W panel 1/2）: -
      |                     ; U7（RP2040搭載Pico W／SC0918）: 3(GND), 8(GND), 13(GND), 18(GND), 23(GND), 28(GND), 33(AGND), 38(GND)
      |                     ; U1（外付けADC／MCP3208-CI/SL）: 8(CH7), 9(DGND), 14(AGND)
      | この場所の直接接続　; P_R8（P_FBからGNDへ接続し、P_R7とともにクランプ電圧設定を構成する／4.99 kΩ）: 2
      | 直接接続の範囲　　　; このラベルから実際の線・分岐・明示的な境界端子だけを追った接続。同名ラベルによる離れた場所への接続はこの欄に含めない。
      | 同一ネット全端子　　; BT1: -
      |                     ; C1: 2(n)
      |                     ; C2: 2(n)
      |                     ; C3: 2(n)
      |                     ; C4: 2(n)
      |                     ; C7: 2(n)
      |                     ; C8: 2(n)
      |                     ; C9: 2(n)
      |                     ; C10: 2(n)
      |                     ; C13: 2(n)
      |                     ; C14: 2(n)
      |                     ; C15: 2(n)
      |                     ; C16: 2(n)
      |                     ; C17: 2
      |                     ; C18: 2
      |                     ; C19: 2
      |                     ; C20: 2
      |                     ; C21: 2
      |                     ; C22: 2
      |                     ; C23: 2
      |                     ; C24: 2
      |                     ; C25: 2
      |                     ; C26: 2
      |                     ; C27: 2
      |                     ; C28: 2
      |                     ; C29: 2
      |                     ; C30: 2
      |                     ; C31: 2
      |                     ; C33: 2
      |                     ; C34: 2
      |                     ; C35: 2
      |                     ; C36: 2
      |                     ; C40: 2
      |                     ; C41: 2
      |                     ; C42: 2
      |                     ; C43: 2
      |                     ; C44: 2
      |                     ; C45: 2
      |                     ; C46: 2
      |                     ; C47: 2
      |                     ; C48: 2
      |                     ; D2: 2(A)
      |                     ; PV1: -
      |                     ; P_CHG: N
      |                     ; P_COUT: N
      |                     ; P_CTMR: N
      |                     ; P_D1: A
      |                     ; P_R3: 2
      |                     ; P_R8: 2
      |                     ; P_RSHDN_PD: 2
      |                     ; P_U1: GND
      |                     ; Q2: 3(S)
      |                     ; Q3: 1(S1), 4(S2)
      |                     ; R1: 2(n)
      |                     ; R18: 2
      |                     ; R21: 2
      |                     ; R24: 2
      |                     ; R35: 2
      |                     ; R42: 2
      |                     ; R44: 2
      |                     ; R48: 2
      |                     ; U1: 8(CH7), 9(DGND), 14(AGND)
      |                     ; U2: 2(GND), 3(REF2), 4(RESERVED_GND)
      |                     ; U3: 2(GND), 3(REF2), 4(RESERVED_GND)
      |                     ; U4: 3(GND)
      |                     ; U5: 3(GND)
      |                     ; U6: 3(GND)
      |                     ; U7: 3(GND), 8(GND), 13(GND), 18(GND), 23(GND), 28(GND), 33(AGND), 38(GND)
      |                     ; U9: 4(VEE)
      |                     ; U10: 1(GNDP), 2(GNDP), 5(GNDP), 8(GNDP), 9(GNDP), 10(GNDP), 11(GNDP), 12(GNDP), 13(GNDP), 14(GNDP), 15(GNDP), 16(GNDP), 17(GNDP), 18(GNDP)
      |                     ; U11: 2(GND)
      |                     ; U12: 2(GND)
      | 接続部品数　　　　　; 72部品（部品番号で集計。同一ネット全体）
      | 接続端子数　　　　　; 99端子（423端子の部品対応表で集計。ラベル・境界ポートの重複は含めない）
      | この場所の端子数　　; 1端子／1部品（同名ラベルによる接続を除く）
      | 同階層同名ラベル数　; 8個（このラベル自身を含む）
      | 全階層の接続ラベル　; 87個（実際に同じノードへつながるラベル。名前が違う別名も含む）
      | 接続ルール　　　　　; 同じ階層の同じラベル名を仮想配線として結ぶ。別のSubsystem内とは名前だけでつながらず、明示的なConnection Portと配線をたどる。色は用途の表示であり接続を決めない。
      | 確認の範囲　　　　　; 現在の保存回路の端子・配線から求めた静的接続。抵抗やICの内部を導線として短絡せずに集計した。説明の更新は動作シミュレーション、タイミング、実部品の性能・実機動作を保証するものではない。
      | 記録の基準　　　　　; measurement_label_layout_20261022_r01/after_layout_graph.json。部品対応表は端子名の対応付けにのみ使用。
      | 
      | 【この説明欄の略語・記号】
      | 用語1　　　　　　　 ; ADC：Analog-to-Digital Converter（アナログ・デジタル変換器）。測定電圧をデジタル値へ変換する回路。電流や温度も、センサーで電圧へ変換した後に読み取る。
      | 用語2　　　　　　　 ; IC：Integrated Circuit（集積回路）。複数の電子素子と機能を小さな半導体チップに集積した部品。
      | 用語3　　　　　　　 ; CH：Channel（測定チャネル）。CH0〜CH7はADCの入力番号であり、同時測定を意味しない。
      | 用語4　　　　　　　 ; MOSFET：Metal-Oxide-Semiconductor Field-Effect Transistor（金属・酸化膜・半導体構造の電界効果トランジスタ）。ゲートとソースの電圧でドレインとソースの導通を制御する素子。N-MOSはNチャネル型を表す。
      | 用語5　　　　　　　 ; LiFePO4：Lithium Iron Phosphate（リン酸鉄リチウム）。電池の正極材料を示す化学式。英語の頭文字を並べた略語ではない。
      | 用語6　　　　　　　 ; GND：Ground（回路の基準電位・電流帰路）。この図の共通基準。保護接地や大地への接続を意味するとは限らない。
      | 用語7　　　　　　　 ; AGND：Analog Ground（アナログ回路の基準端子）。アナログ部分の電流帰路。現図では共通GNDへ接続されるが、実装時の電流経路への配慮は別途必要。
      | 用語8　　　　　　　 ; DGND：Digital Ground（デジタル回路の基準端子）。デジタル部分の電流帰路。現図では共通GNDへ接続される。
      | 用語9　　　　　　　 ; FB：Feedback（帰還）。出力などを検出して内部制御へ戻すための信号・端子。
      | 用語10　　　　　　　; VREF/REF：基準電圧を表す端子名。REFはReference（基準）の意味。ADCの変換尺度や電流アンプの出力基準に使う。REF1/REF2の接続電位は個別に確認する。
      | 用語11　　　　　　　; VCC/VDD/VEE/VS：ICの電源端子名。文字の歴史的な由来を現在の接続機能へ当てはめない。現回路のVEEはU8/U10では浮動基準SW、U9ではGND。各電圧・基準は端子と接続を参照する。
      | 用語12　　　　　　　; GNDP：U10の一次側電源の基準端子。絶縁電源の入力側GND。二次側基準VEE=SWと直接同一の導体ではない。
      | 用語13　　　　　　　; SW：Switching Node（スイッチング点）。主電力段の上下MOSFETとL1がつながる、電圧が高速に切り替わる点。GNDとは別電位。
      | 用語14　　　　　　　; PROT_RETURN：保護回路の共通帰路。PROTはProtection（保護）、RETURNは帰路。プロトタイプの略ではなく、現回路では共通GNDへつながる。
  RETURN_label_4 : ConnectionLabel  Description=|  Label=PROT_RETURN
      | この回路での名前　　; PROT_RETURN
      | 種別　　　　　　　　; ConnectionLabel
      | この回路での役割　　; 保護回路の帰路を、外側の共通GNDへ結ぶ。このラベルはプロトタイプという意味ではなく保護回路の戻り線を示す。明示的な境界端子を経由してBT1負極・PV1負極と同じノードになる。
      | 共通帰路の代表接続　; P_U1（保護MOSFETを制御する保護IC／LTC4364IMS-1#PBF）: GND
      |                     ; BT1（充電先の蓄電池／51.2V 100Ah LiFePO4）: -
      |                     ; PV1（直列太陽電池列の負極側パネル／400W panel 1/2）: -
      |                     ; U7（RP2040搭載Pico W／SC0918）: 3(GND), 8(GND), 13(GND), 18(GND), 23(GND), 28(GND), 33(AGND), 38(GND)
      |                     ; U1（外付けADC／MCP3208-CI/SL）: 8(CH7), 9(DGND), 14(AGND)
      | この場所の直接接続　; P_COUT（保護回路出力側のコンデンサ／330 µF）: N
      | 直接接続の範囲　　　; このラベルから実際の線・分岐・明示的な境界端子だけを追った接続。同名ラベルによる離れた場所への接続はこの欄に含めない。
      | 同一ネット全端子　　; BT1: -
      |                     ; C1: 2(n)
      |                     ; C2: 2(n)
      |                     ; C3: 2(n)
      |                     ; C4: 2(n)
      |                     ; C7: 2(n)
      |                     ; C8: 2(n)
      |                     ; C9: 2(n)
      |                     ; C10: 2(n)
      |                     ; C13: 2(n)
      |                     ; C14: 2(n)
      |                     ; C15: 2(n)
      |                     ; C16: 2(n)
      |                     ; C17: 2
      |                     ; C18: 2
      |                     ; C19: 2
      |                     ; C20: 2
      |                     ; C21: 2
      |                     ; C22: 2
      |                     ; C23: 2
      |                     ; C24: 2
      |                     ; C25: 2
      |                     ; C26: 2
      |                     ; C27: 2
      |                     ; C28: 2
      |                     ; C29: 2
      |                     ; C30: 2
      |                     ; C31: 2
      |                     ; C33: 2
      |                     ; C34: 2
      |                     ; C35: 2
      |                     ; C36: 2
      |                     ; C40: 2
      |                     ; C41: 2
      |                     ; C42: 2
      |                     ; C43: 2
      |                     ; C44: 2
      |                     ; C45: 2
      |                     ; C46: 2
      |                     ; C47: 2
      |                     ; C48: 2
      |                     ; D2: 2(A)
      |                     ; PV1: -
      |                     ; P_CHG: N
      |                     ; P_COUT: N
      |                     ; P_CTMR: N
      |                     ; P_D1: A
      |                     ; P_R3: 2
      |                     ; P_R8: 2
      |                     ; P_RSHDN_PD: 2
      |                     ; P_U1: GND
      |                     ; Q2: 3(S)
      |                     ; Q3: 1(S1), 4(S2)
      |                     ; R1: 2(n)
      |                     ; R18: 2
      |                     ; R21: 2
      |                     ; R24: 2
      |                     ; R35: 2
      |                     ; R42: 2
      |                     ; R44: 2
      |                     ; R48: 2
      |                     ; U1: 8(CH7), 9(DGND), 14(AGND)
      |                     ; U2: 2(GND), 3(REF2), 4(RESERVED_GND)
      |                     ; U3: 2(GND), 3(REF2), 4(RESERVED_GND)
      |                     ; U4: 3(GND)
      |                     ; U5: 3(GND)
      |                     ; U6: 3(GND)
      |                     ; U7: 3(GND), 8(GND), 13(GND), 18(GND), 23(GND), 28(GND), 33(AGND), 38(GND)
      |                     ; U9: 4(VEE)
      |                     ; U10: 1(GNDP), 2(GNDP), 5(GNDP), 8(GNDP), 9(GNDP), 10(GNDP), 11(GNDP), 12(GNDP), 13(GNDP), 14(GNDP), 15(GNDP), 16(GNDP), 17(GNDP), 18(GNDP)
      |                     ; U11: 2(GND)
      |                     ; U12: 2(GND)
      | 接続部品数　　　　　; 72部品（部品番号で集計。同一ネット全体）
      | 接続端子数　　　　　; 99端子（423端子の部品対応表で集計。ラベル・境界ポートの重複は含めない）
      | この場所の端子数　　; 1端子／1部品（同名ラベルによる接続を除く）
      | 同階層同名ラベル数　; 8個（このラベル自身を含む）
      | 全階層の接続ラベル　; 87個（実際に同じノードへつながるラベル。名前が違う別名も含む）
      | 接続ルール　　　　　; 同じ階層の同じラベル名を仮想配線として結ぶ。別のSubsystem内とは名前だけでつながらず、明示的なConnection Portと配線をたどる。色は用途の表示であり接続を決めない。
      | 確認の範囲　　　　　; 現在の保存回路の端子・配線から求めた静的接続。抵抗やICの内部を導線として短絡せずに集計した。説明の更新は動作シミュレーション、タイミング、実部品の性能・実機動作を保証するものではない。
      | 記録の基準　　　　　; measurement_label_layout_20261022_r01/after_layout_graph.json。部品対応表は端子名の対応付けにのみ使用。
      | 
      | 【この説明欄の略語・記号】
      | 用語1　　　　　　　 ; ADC：Analog-to-Digital Converter（アナログ・デジタル変換器）。測定電圧をデジタル値へ変換する回路。電流や温度も、センサーで電圧へ変換した後に読み取る。
      | 用語2　　　　　　　 ; IC：Integrated Circuit（集積回路）。複数の電子素子と機能を小さな半導体チップに集積した部品。
      | 用語3　　　　　　　 ; CH：Channel（測定チャネル）。CH0〜CH7はADCの入力番号であり、同時測定を意味しない。
      | 用語4　　　　　　　 ; MOSFET：Metal-Oxide-Semiconductor Field-Effect Transistor（金属・酸化膜・半導体構造の電界効果トランジスタ）。ゲートとソースの電圧でドレインとソースの導通を制御する素子。N-MOSはNチャネル型を表す。
      | 用語5　　　　　　　 ; LiFePO4：Lithium Iron Phosphate（リン酸鉄リチウム）。電池の正極材料を示す化学式。英語の頭文字を並べた略語ではない。
      | 用語6　　　　　　　 ; GND：Ground（回路の基準電位・電流帰路）。この図の共通基準。保護接地や大地への接続を意味するとは限らない。
      | 用語7　　　　　　　 ; AGND：Analog Ground（アナログ回路の基準端子）。アナログ部分の電流帰路。現図では共通GNDへ接続されるが、実装時の電流経路への配慮は別途必要。
      | 用語8　　　　　　　 ; DGND：Digital Ground（デジタル回路の基準端子）。デジタル部分の電流帰路。現図では共通GNDへ接続される。
      | 用語9　　　　　　　 ; VREF/REF：基準電圧を表す端子名。REFはReference（基準）の意味。ADCの変換尺度や電流アンプの出力基準に使う。REF1/REF2の接続電位は個別に確認する。
      | 用語10　　　　　　　; VCC/VDD/VEE/VS：ICの電源端子名。文字の歴史的な由来を現在の接続機能へ当てはめない。現回路のVEEはU8/U10では浮動基準SW、U9ではGND。各電圧・基準は端子と接続を参照する。
      | 用語11　　　　　　　; GNDP：U10の一次側電源の基準端子。絶縁電源の入力側GND。二次側基準VEE=SWと直接同一の導体ではない。
      | 用語12　　　　　　　; SW：Switching Node（スイッチング点）。主電力段の上下MOSFETとL1がつながる、電圧が高速に切り替わる点。GNDとは別電位。
      | 用語13　　　　　　　; PROT_RETURN：保護回路の共通帰路。PROTはProtection（保護）、RETURNは帰路。プロトタイプの略ではなく、現回路では共通GNDへつながる。
  RETURN_label_5 : ConnectionLabel  Description=|  Label=PROT_RETURN
      | この回路での名前　　; PROT_RETURN
      | 種別　　　　　　　　; ConnectionLabel
      | この回路での役割　　; 保護回路の帰路を、外側の共通GNDへ結ぶ。このラベルはプロトタイプという意味ではなく保護回路の戻り線を示す。明示的な境界端子を経由してBT1負極・PV1負極と同じノードになる。
      | 共通帰路の代表接続　; P_U1（保護MOSFETを制御する保護IC／LTC4364IMS-1#PBF）: GND
      |                     ; BT1（充電先の蓄電池／51.2V 100Ah LiFePO4）: -
      |                     ; PV1（直列太陽電池列の負極側パネル／400W panel 1/2）: -
      |                     ; U7（RP2040搭載Pico W／SC0918）: 3(GND), 8(GND), 13(GND), 18(GND), 23(GND), 28(GND), 33(AGND), 38(GND)
      |                     ; U1（外付けADC／MCP3208-CI/SL）: 8(CH7), 9(DGND), 14(AGND)
      | この場所の直接接続　; P_CTMR（TMR–GND間に置き、故障継続時間の積算・遮断タイミングへ関与させる／100 nF）: N
      | 直接接続の範囲　　　; このラベルから実際の線・分岐・明示的な境界端子だけを追った接続。同名ラベルによる離れた場所への接続はこの欄に含めない。
      | 同一ネット全端子　　; BT1: -
      |                     ; C1: 2(n)
      |                     ; C2: 2(n)
      |                     ; C3: 2(n)
      |                     ; C4: 2(n)
      |                     ; C7: 2(n)
      |                     ; C8: 2(n)
      |                     ; C9: 2(n)
      |                     ; C10: 2(n)
      |                     ; C13: 2(n)
      |                     ; C14: 2(n)
      |                     ; C15: 2(n)
      |                     ; C16: 2(n)
      |                     ; C17: 2
      |                     ; C18: 2
      |                     ; C19: 2
      |                     ; C20: 2
      |                     ; C21: 2
      |                     ; C22: 2
      |                     ; C23: 2
      |                     ; C24: 2
      |                     ; C25: 2
      |                     ; C26: 2
      |                     ; C27: 2
      |                     ; C28: 2
      |                     ; C29: 2
      |                     ; C30: 2
      |                     ; C31: 2
      |                     ; C33: 2
      |                     ; C34: 2
      |                     ; C35: 2
      |                     ; C36: 2
      |                     ; C40: 2
      |                     ; C41: 2
      |                     ; C42: 2
      |                     ; C43: 2
      |                     ; C44: 2
      |                     ; C45: 2
      |                     ; C46: 2
      |                     ; C47: 2
      |                     ; C48: 2
      |                     ; D2: 2(A)
      |                     ; PV1: -
      |                     ; P_CHG: N
      |                     ; P_COUT: N
      |                     ; P_CTMR: N
      |                     ; P_D1: A
      |                     ; P_R3: 2
      |                     ; P_R8: 2
      |                     ; P_RSHDN_PD: 2
      |                     ; P_U1: GND
      |                     ; Q2: 3(S)
      |                     ; Q3: 1(S1), 4(S2)
      |                     ; R1: 2(n)
      |                     ; R18: 2
      |                     ; R21: 2
      |                     ; R24: 2
      |                     ; R35: 2
      |                     ; R42: 2
      |                     ; R44: 2
      |                     ; R48: 2
      |                     ; U1: 8(CH7), 9(DGND), 14(AGND)
      |                     ; U2: 2(GND), 3(REF2), 4(RESERVED_GND)
      |                     ; U3: 2(GND), 3(REF2), 4(RESERVED_GND)
      |                     ; U4: 3(GND)
      |                     ; U5: 3(GND)
      |                     ; U6: 3(GND)
      |                     ; U7: 3(GND), 8(GND), 13(GND), 18(GND), 23(GND), 28(GND), 33(AGND), 38(GND)
      |                     ; U9: 4(VEE)
      |                     ; U10: 1(GNDP), 2(GNDP), 5(GNDP), 8(GNDP), 9(GNDP), 10(GNDP), 11(GNDP), 12(GNDP), 13(GNDP), 14(GNDP), 15(GNDP), 16(GNDP), 17(GNDP), 18(GNDP)
      |                     ; U11: 2(GND)
      |                     ; U12: 2(GND)
      | 接続部品数　　　　　; 72部品（部品番号で集計。同一ネット全体）
      | 接続端子数　　　　　; 99端子（423端子の部品対応表で集計。ラベル・境界ポートの重複は含めない）
      | この場所の端子数　　; 1端子／1部品（同名ラベルによる接続を除く）
      | 同階層同名ラベル数　; 8個（このラベル自身を含む）
      | 全階層の接続ラベル　; 87個（実際に同じノードへつながるラベル。名前が違う別名も含む）
      | 接続ルール　　　　　; 同じ階層の同じラベル名を仮想配線として結ぶ。別のSubsystem内とは名前だけでつながらず、明示的なConnection Portと配線をたどる。色は用途の表示であり接続を決めない。
      | 確認の範囲　　　　　; 現在の保存回路の端子・配線から求めた静的接続。抵抗やICの内部を導線として短絡せずに集計した。説明の更新は動作シミュレーション、タイミング、実部品の性能・実機動作を保証するものではない。
      | 記録の基準　　　　　; measurement_label_layout_20261022_r01/after_layout_graph.json。部品対応表は端子名の対応付けにのみ使用。
      | 
      | 【この説明欄の略語・記号】
      | 用語1　　　　　　　 ; ADC：Analog-to-Digital Converter（アナログ・デジタル変換器）。測定電圧をデジタル値へ変換する回路。電流や温度も、センサーで電圧へ変換した後に読み取る。
      | 用語2　　　　　　　 ; IC：Integrated Circuit（集積回路）。複数の電子素子と機能を小さな半導体チップに集積した部品。
      | 用語3　　　　　　　 ; CH：Channel（測定チャネル）。CH0〜CH7はADCの入力番号であり、同時測定を意味しない。
      | 用語4　　　　　　　 ; MOSFET：Metal-Oxide-Semiconductor Field-Effect Transistor（金属・酸化膜・半導体構造の電界効果トランジスタ）。ゲートとソースの電圧でドレインとソースの導通を制御する素子。N-MOSはNチャネル型を表す。
      | 用語5　　　　　　　 ; LiFePO4：Lithium Iron Phosphate（リン酸鉄リチウム）。電池の正極材料を示す化学式。英語の頭文字を並べた略語ではない。
      | 用語6　　　　　　　 ; GND：Ground（回路の基準電位・電流帰路）。この図の共通基準。保護接地や大地への接続を意味するとは限らない。
      | 用語7　　　　　　　 ; AGND：Analog Ground（アナログ回路の基準端子）。アナログ部分の電流帰路。現図では共通GNDへ接続されるが、実装時の電流経路への配慮は別途必要。
      | 用語8　　　　　　　 ; DGND：Digital Ground（デジタル回路の基準端子）。デジタル部分の電流帰路。現図では共通GNDへ接続される。
      | 用語9　　　　　　　 ; TMR：Timer（時間設定端子）。LTC4364では外付けコンデンサにより故障継続時間の判定などに関係する時間を設定する。
      | 用語10　　　　　　　; VREF/REF：基準電圧を表す端子名。REFはReference（基準）の意味。ADCの変換尺度や電流アンプの出力基準に使う。REF1/REF2の接続電位は個別に確認する。
      | 用語11　　　　　　　; VCC/VDD/VEE/VS：ICの電源端子名。文字の歴史的な由来を現在の接続機能へ当てはめない。現回路のVEEはU8/U10では浮動基準SW、U9ではGND。各電圧・基準は端子と接続を参照する。
      | 用語12　　　　　　　; GNDP：U10の一次側電源の基準端子。絶縁電源の入力側GND。二次側基準VEE=SWと直接同一の導体ではない。
      | 用語13　　　　　　　; SW：Switching Node（スイッチング点）。主電力段の上下MOSFETとL1がつながる、電圧が高速に切り替わる点。GNDとは別電位。
      | 用語14　　　　　　　; PROT_RETURN：保護回路の共通帰路。PROTはProtection（保護）、RETURNは帰路。プロトタイプの略ではなく、現回路では共通GNDへつながる。
  RETURN_label_6 : ConnectionLabel  Description=|  Label=PROT_RETURN
      | この回路での名前　　; PROT_RETURN
      | 種別　　　　　　　　; ConnectionLabel
      | この回路での役割　　; 保護回路の帰路を、外側の共通GNDへ結ぶ。このラベルはプロトタイプという意味ではなく保護回路の戻り線を示す。明示的な境界端子を経由してBT1負極・PV1負極と同じノードになる。
      | 共通帰路の代表接続　; P_U1（保護MOSFETを制御する保護IC／LTC4364IMS-1#PBF）: GND
      |                     ; BT1（充電先の蓄電池／51.2V 100Ah LiFePO4）: -
      |                     ; PV1（直列太陽電池列の負極側パネル／400W panel 1/2）: -
      |                     ; U7（RP2040搭載Pico W／SC0918）: 3(GND), 8(GND), 13(GND), 18(GND), 23(GND), 28(GND), 33(AGND), 38(GND)
      |                     ; U1（外付けADC／MCP3208-CI/SL）: 8(CH7), 9(DGND), 14(AGND)
      | この場所の直接接続　; P_D1（P_VCC–GND間でLTC4364の電源電圧上昇を抑える／68 V）: A
      | 直接接続の範囲　　　; このラベルから実際の線・分岐・明示的な境界端子だけを追った接続。同名ラベルによる離れた場所への接続はこの欄に含めない。
      | 同一ネット全端子　　; BT1: -
      |                     ; C1: 2(n)
      |                     ; C2: 2(n)
      |                     ; C3: 2(n)
      |                     ; C4: 2(n)
      |                     ; C7: 2(n)
      |                     ; C8: 2(n)
      |                     ; C9: 2(n)
      |                     ; C10: 2(n)
      |                     ; C13: 2(n)
      |                     ; C14: 2(n)
      |                     ; C15: 2(n)
      |                     ; C16: 2(n)
      |                     ; C17: 2
      |                     ; C18: 2
      |                     ; C19: 2
      |                     ; C20: 2
      |                     ; C21: 2
      |                     ; C22: 2
      |                     ; C23: 2
      |                     ; C24: 2
      |                     ; C25: 2
      |                     ; C26: 2
      |                     ; C27: 2
      |                     ; C28: 2
      |                     ; C29: 2
      |                     ; C30: 2
      |                     ; C31: 2
      |                     ; C33: 2
      |                     ; C34: 2
      |                     ; C35: 2
      |                     ; C36: 2
      |                     ; C40: 2
      |                     ; C41: 2
      |                     ; C42: 2
      |                     ; C43: 2
      |                     ; C44: 2
      |                     ; C45: 2
      |                     ; C46: 2
      |                     ; C47: 2
      |                     ; C48: 2
      |                     ; D2: 2(A)
      |                     ; PV1: -
      |                     ; P_CHG: N
      |                     ; P_COUT: N
      |                     ; P_CTMR: N
      |                     ; P_D1: A
      |                     ; P_R3: 2
      |                     ; P_R8: 2
      |                     ; P_RSHDN_PD: 2
      |                     ; P_U1: GND
      |                     ; Q2: 3(S)
      |                     ; Q3: 1(S1), 4(S2)
      |                     ; R1: 2(n)
      |                     ; R18: 2
      |                     ; R21: 2
      |                     ; R24: 2
      |                     ; R35: 2
      |                     ; R42: 2
      |                     ; R44: 2
      |                     ; R48: 2
      |                     ; U1: 8(CH7), 9(DGND), 14(AGND)
      |                     ; U2: 2(GND), 3(REF2), 4(RESERVED_GND)
      |                     ; U3: 2(GND), 3(REF2), 4(RESERVED_GND)
      |                     ; U4: 3(GND)
      |                     ; U5: 3(GND)
      |                     ; U6: 3(GND)
      |                     ; U7: 3(GND), 8(GND), 13(GND), 18(GND), 23(GND), 28(GND), 33(AGND), 38(GND)
      |                     ; U9: 4(VEE)
      |                     ; U10: 1(GNDP), 2(GNDP), 5(GNDP), 8(GNDP), 9(GNDP), 10(GNDP), 11(GNDP), 12(GNDP), 13(GNDP), 14(GNDP), 15(GNDP), 16(GNDP), 17(GNDP), 18(GNDP)
      |                     ; U11: 2(GND)
      |                     ; U12: 2(GND)
      | 接続部品数　　　　　; 72部品（部品番号で集計。同一ネット全体）
      | 接続端子数　　　　　; 99端子（423端子の部品対応表で集計。ラベル・境界ポートの重複は含めない）
      | この場所の端子数　　; 1端子／1部品（同名ラベルによる接続を除く）
      | 同階層同名ラベル数　; 8個（このラベル自身を含む）
      | 全階層の接続ラベル　; 87個（実際に同じノードへつながるラベル。名前が違う別名も含む）
      | 接続ルール　　　　　; 同じ階層の同じラベル名を仮想配線として結ぶ。別のSubsystem内とは名前だけでつながらず、明示的なConnection Portと配線をたどる。色は用途の表示であり接続を決めない。
      | 確認の範囲　　　　　; 現在の保存回路の端子・配線から求めた静的接続。抵抗やICの内部を導線として短絡せずに集計した。説明の更新は動作シミュレーション、タイミング、実部品の性能・実機動作を保証するものではない。
      | 記録の基準　　　　　; measurement_label_layout_20261022_r01/after_layout_graph.json。部品対応表は端子名の対応付けにのみ使用。
      | 
      | 【この説明欄の略語・記号】
      | 用語1　　　　　　　 ; ADC：Analog-to-Digital Converter（アナログ・デジタル変換器）。測定電圧をデジタル値へ変換する回路。電流や温度も、センサーで電圧へ変換した後に読み取る。
      | 用語2　　　　　　　 ; IC：Integrated Circuit（集積回路）。複数の電子素子と機能を小さな半導体チップに集積した部品。
      | 用語3　　　　　　　 ; CH：Channel（測定チャネル）。CH0〜CH7はADCの入力番号であり、同時測定を意味しない。
      | 用語4　　　　　　　 ; MOSFET：Metal-Oxide-Semiconductor Field-Effect Transistor（金属・酸化膜・半導体構造の電界効果トランジスタ）。ゲートとソースの電圧でドレインとソースの導通を制御する素子。N-MOSはNチャネル型を表す。
      | 用語5　　　　　　　 ; LiFePO4：Lithium Iron Phosphate（リン酸鉄リチウム）。電池の正極材料を示す化学式。英語の頭文字を並べた略語ではない。
      | 用語6　　　　　　　 ; GND：Ground（回路の基準電位・電流帰路）。この図の共通基準。保護接地や大地への接続を意味するとは限らない。
      | 用語7　　　　　　　 ; AGND：Analog Ground（アナログ回路の基準端子）。アナログ部分の電流帰路。現図では共通GNDへ接続されるが、実装時の電流経路への配慮は別途必要。
      | 用語8　　　　　　　 ; DGND：Digital Ground（デジタル回路の基準端子）。デジタル部分の電流帰路。現図では共通GNDへ接続される。
      | 用語9　　　　　　　 ; VREF/REF：基準電圧を表す端子名。REFはReference（基準）の意味。ADCの変換尺度や電流アンプの出力基準に使う。REF1/REF2の接続電位は個別に確認する。
      | 用語10　　　　　　　; VCC/VDD/VEE/VS：ICの電源端子名。文字の歴史的な由来を現在の接続機能へ当てはめない。現回路のVEEはU8/U10では浮動基準SW、U9ではGND。各電圧・基準は端子と接続を参照する。
      | 用語11　　　　　　　; GNDP：U10の一次側電源の基準端子。絶縁電源の入力側GND。二次側基準VEE=SWと直接同一の導体ではない。
      | 用語12　　　　　　　; SW：Switching Node（スイッチング点）。主電力段の上下MOSFETとL1がつながる、電圧が高速に切り替わる点。GNDとは別電位。
      | 用語13　　　　　　　; PROT_RETURN：保護回路の共通帰路。PROTはProtection（保護）、RETURNは帰路。プロトタイプの略ではなく、現回路では共通GNDへつながる。
  RETURN_label_7 : ConnectionLabel  Description=|  Label=PROT_RETURN
      | この回路での名前　　; PROT_RETURN
      | 種別　　　　　　　　; ConnectionLabel
      | この回路での役割　　; 保護回路の帰路を、外側の共通GNDへ結ぶ。このラベルはプロトタイプという意味ではなく保護回路の戻り線を示す。明示的な境界端子を経由してBT1負極・PV1負極と同じノードになる。
      | 共通帰路の代表接続　; P_U1（保護MOSFETを制御する保護IC／LTC4364IMS-1#PBF）: GND
      |                     ; BT1（充電先の蓄電池／51.2V 100Ah LiFePO4）: -
      |                     ; PV1（直列太陽電池列の負極側パネル／400W panel 1/2）: -
      |                     ; U7（RP2040搭載Pico W／SC0918）: 3(GND), 8(GND), 13(GND), 18(GND), 23(GND), 28(GND), 33(AGND), 38(GND)
      |                     ; U1（外付けADC／MCP3208-CI/SL）: 8(CH7), 9(DGND), 14(AGND)
      | この場所の直接接続　; P_CHG（HGATE–GND間へ置き、P_Q1起動時のゲート電圧変化と制御応答に関与させる／47 nF）: N
      | 直接接続の範囲　　　; このラベルから実際の線・分岐・明示的な境界端子だけを追った接続。同名ラベルによる離れた場所への接続はこの欄に含めない。
      | 同一ネット全端子　　; BT1: -
      |                     ; C1: 2(n)
      |                     ; C2: 2(n)
      |                     ; C3: 2(n)
      |                     ; C4: 2(n)
      |                     ; C7: 2(n)
      |                     ; C8: 2(n)
      |                     ; C9: 2(n)
      |                     ; C10: 2(n)
      |                     ; C13: 2(n)
      |                     ; C14: 2(n)
      |                     ; C15: 2(n)
      |                     ; C16: 2(n)
      |                     ; C17: 2
      |                     ; C18: 2
      |                     ; C19: 2
      |                     ; C20: 2
      |                     ; C21: 2
      |                     ; C22: 2
      |                     ; C23: 2
      |                     ; C24: 2
      |                     ; C25: 2
      |                     ; C26: 2
      |                     ; C27: 2
      |                     ; C28: 2
      |                     ; C29: 2
      |                     ; C30: 2
      |                     ; C31: 2
      |                     ; C33: 2
      |                     ; C34: 2
      |                     ; C35: 2
      |                     ; C36: 2
      |                     ; C40: 2
      |                     ; C41: 2
      |                     ; C42: 2
      |                     ; C43: 2
      |                     ; C44: 2
      |                     ; C45: 2
      |                     ; C46: 2
      |                     ; C47: 2
      |                     ; C48: 2
      |                     ; D2: 2(A)
      |                     ; PV1: -
      |                     ; P_CHG: N
      |                     ; P_COUT: N
      |                     ; P_CTMR: N
      |                     ; P_D1: A
      |                     ; P_R3: 2
      |                     ; P_R8: 2
      |                     ; P_RSHDN_PD: 2
      |                     ; P_U1: GND
      |                     ; Q2: 3(S)
      |                     ; Q3: 1(S1), 4(S2)
      |                     ; R1: 2(n)
      |                     ; R18: 2
      |                     ; R21: 2
      |                     ; R24: 2
      |                     ; R35: 2
      |                     ; R42: 2
      |                     ; R44: 2
      |                     ; R48: 2
      |                     ; U1: 8(CH7), 9(DGND), 14(AGND)
      |                     ; U2: 2(GND), 3(REF2), 4(RESERVED_GND)
      |                     ; U3: 2(GND), 3(REF2), 4(RESERVED_GND)
      |                     ; U4: 3(GND)
      |                     ; U5: 3(GND)
      |                     ; U6: 3(GND)
      |                     ; U7: 3(GND), 8(GND), 13(GND), 18(GND), 23(GND), 28(GND), 33(AGND), 38(GND)
      |                     ; U9: 4(VEE)
      |                     ; U10: 1(GNDP), 2(GNDP), 5(GNDP), 8(GNDP), 9(GNDP), 10(GNDP), 11(GNDP), 12(GNDP), 13(GNDP), 14(GNDP), 15(GNDP), 16(GNDP), 17(GNDP), 18(GNDP)
      |                     ; U11: 2(GND)
      |                     ; U12: 2(GND)
      | 接続部品数　　　　　; 72部品（部品番号で集計。同一ネット全体）
      | 接続端子数　　　　　; 99端子（423端子の部品対応表で集計。ラベル・境界ポートの重複は含めない）
      | この場所の端子数　　; 1端子／1部品（同名ラベルによる接続を除く）
      | 同階層同名ラベル数　; 8個（このラベル自身を含む）
      | 全階層の接続ラベル　; 87個（実際に同じノードへつながるラベル。名前が違う別名も含む）
      | 接続ルール　　　　　; 同じ階層の同じラベル名を仮想配線として結ぶ。別のSubsystem内とは名前だけでつながらず、明示的なConnection Portと配線をたどる。色は用途の表示であり接続を決めない。
      | 確認の範囲　　　　　; 現在の保存回路の端子・配線から求めた静的接続。抵抗やICの内部を導線として短絡せずに集計した。説明の更新は動作シミュレーション、タイミング、実部品の性能・実機動作を保証するものではない。
      | 記録の基準　　　　　; measurement_label_layout_20261022_r01/after_layout_graph.json。部品対応表は端子名の対応付けにのみ使用。
      | 
      | 【この説明欄の略語・記号】
      | 用語1　　　　　　　 ; ADC：Analog-to-Digital Converter（アナログ・デジタル変換器）。測定電圧をデジタル値へ変換する回路。電流や温度も、センサーで電圧へ変換した後に読み取る。
      | 用語2　　　　　　　 ; IC：Integrated Circuit（集積回路）。複数の電子素子と機能を小さな半導体チップに集積した部品。
      | 用語3　　　　　　　 ; PWM：Pulse Width Modulation（パルス幅変調）。周期に対するON時間の割合を変えて、スイッチの平均的な電力伝達を調整する方式。
      | 用語4　　　　　　　 ; CH：Channel（測定チャネル）。CH0〜CH7はADCの入力番号であり、同時測定を意味しない。
      | 用語5　　　　　　　 ; MOSFET：Metal-Oxide-Semiconductor Field-Effect Transistor（金属・酸化膜・半導体構造の電界効果トランジスタ）。ゲートとソースの電圧でドレインとソースの導通を制御する素子。N-MOSはNチャネル型を表す。
      | 用語6　　　　　　　 ; LiFePO4：Lithium Iron Phosphate（リン酸鉄リチウム）。電池の正極材料を示す化学式。英語の頭文字を並べた略語ではない。
      | 用語7　　　　　　　 ; GND：Ground（回路の基準電位・電流帰路）。この図の共通基準。保護接地や大地への接続を意味するとは限らない。
      | 用語8　　　　　　　 ; AGND：Analog Ground（アナログ回路の基準端子）。アナログ部分の電流帰路。現図では共通GNDへ接続されるが、実装時の電流経路への配慮は別途必要。
      | 用語9　　　　　　　 ; DGND：Digital Ground（デジタル回路の基準端子）。デジタル部分の電流帰路。現図では共通GNDへ接続される。
      | 用語10　　　　　　　; VREF/REF：基準電圧を表す端子名。REFはReference（基準）の意味。ADCの変換尺度や電流アンプの出力基準に使う。REF1/REF2の接続電位は個別に確認する。
      | 用語11　　　　　　　; VCC/VDD/VEE/VS：ICの電源端子名。文字の歴史的な由来を現在の接続機能へ当てはめない。現回路のVEEはU8/U10では浮動基準SW、U9ではGND。各電圧・基準は端子と接続を参照する。
      | 用語12　　　　　　　; GNDP：U10の一次側電源の基準端子。絶縁電源の入力側GND。二次側基準VEE=SWと直接同一の導体ではない。
      | 用語13　　　　　　　; HGATE/DGATE：LTC4364の二つの外付けMOSFETゲート駆動出力。HGATEは主に電圧・電流制限側のP_Q1、DGATEは理想ダイオード／逆流防止側のP_Q2を駆動する。主電力段の上下PWMとは別の仕組み。
      | 用語14　　　　　　　; SW：Switching Node（スイッチング点）。主電力段の上下MOSFETとL1がつながる、電圧が高速に切り替わる点。GNDとは別電位。
      | 用語15　　　　　　　; PROT_RETURN：保護回路の共通帰路。PROTはProtection（保護）、RETURNは帰路。プロトタイプの略ではなく、現回路では共通GNDへつながる。
  RSNS_10mOhm : fl_lib/Electrical/Electrical Elements/Resistor  Description=|  R=0.0027 Ohm  i_specify=off  i_priority=None  i=0 A  i_nominal_specify=off  i_nominal_value=1  i_nominal_unit=A  v_specify=off  v_priority=None  v=0 V  v_nominal_specify=off  v_nominal_value=1  v_nominal_unit=V
      | この回路での名前　　; P_RSNS
      | 部品名　　　　　　　; WSL36372L700FEA
      | この回路での役割　　; 保護IC LTC4364が、蓄電池へ流れる電流を制限するための判断に使う、小さな抵抗。
      | ここでの動き　　　　; 充電経路に入れた2.7 mΩに電流が流れると、電流に比例した微小な電圧差が生まれる。LTC4364はその差を読み、電流制限に用いる。マイコンの通常測定用R2・R27とは別の保護用検出経路で、実部品では電力端子と測定端子を分けて配線する。
      | 
      | 【詳しい働き・仕様・接続・確認の範囲】
      | 部品種別　　　　　　; 保護用電流制限シャント
      | 公称値　　　　　　　; 2.7 mΩ
      | 配置目的　　　　　　; P_SENSE–BAT_PLUS間の電圧差をLTC4364へ渡し、電流制限の判断量を作る。
      | 意図する動作　　　　; 2.7 mΩ。通常測定用R2/R27とは別の保護経路。実部品は4端子Kelvin品であり、図面の2端子集中表現はPCBの電流端子と検出端子を短絡配線してよい意味ではない。
      | 端子と接続　　　　　; 1 1 → P_SENSE、2 2 → BAT_PLUS
      | 公称値の公差　　　　; ±1%（既存部品資料の値）
      | 部品資料の根拠　　　; Vishay WSL3637データシート30099の2.7 mΩ・1%・4端子シリーズと、メーカーPCNに記載されたWSL36372L700FEAとの既存照合記録。
      | モデルの範囲　　　　; Simscape抵抗の集中定数表現。部品の許容差、定格電力、温度係数、寄生インダクタンスの適合を示すものではない。
      | モデル設定　　　　　; R=2.7 mΩ。これらは保存モデルの設定値であり、すべてが実部品の保証値という意味ではない。
      | 確認の範囲　　　　　; 本説明は保存回路の部品情報・端子割当・既存設計意図を整理したもの。今回の説明更新によって新たな動作試験や実機検証を実施した意味ではない。
      | 設計記録　　　　　　; evaluation\component_annotations_20261022_r01\before_graph.json
      | evaluation\component_annotations_20261022_r01\before_metadata.json
      | evaluation\protection_capacitor_integration_20261021_r01\final_delivery\independent_readback\physical_bom.json
      | evaluation\protection_capacitor_integration_20261021_r01\protection_review\component_net_map.json
      | 
      | 【この説明欄の略語・記号】
      | 用語1　　　　　　　 ; PCB：Printed Circuit Board（プリント配線板）。部品を実装し、銅配線で接続する基板。
      | 用語2　　　　　　　 ; PCN：Product Change Notification（製品変更通知）。メーカーが仕様・製造などの変更を知らせる文書。部品の採用・動作保証そのものではない。
  R_EN_SERIES_1k : fl_lib/Electrical/Electrical Elements/Resistor  Description=|  R=1000 Ohm  i_specify=off  i_priority=None  i=0 A  i_nominal_specify=off  i_nominal_value=1  i_nominal_unit=A  v_specify=off  v_priority=None  v=0 V  v_nominal_specify=off  v_nominal_value=1  v_nominal_unit=V
      | この回路での名前　　; P_RSHDN_SER
      | 部品名　　　　　　　; CRCW08051K00FKEA
      | この回路での役割　　; マイコンから保護IC LTC4364へ、主電力経路の動作許可・停止の指令を伝える接続に入れた抵抗。
      | ここでの動き　　　　; マイコンのMAIN_ENと保護ICのSHDNの間に1 kΩを置く。P_RSHDN_PDと組み合わせて、マイコンが信号を出すときと端子が開放されるときの入力電圧を決める。IC側の内部プルアップも含めて扱う。
      | 
      | 【詳しい働き・仕様・接続・確認の範囲】
      | 部品種別　　　　　　; 停止制御入力の直列抵抗
      | 公称値　　　　　　　; 1 kΩ
      | 配置目的　　　　　　; RP2040のMAIN_ENとLTC4364のSHDN間へ入る。
      | 意図する動作　　　　; P_RSHDN_PDと組み合わせ、MCU駆動時とHi-Z時のSHDN電圧を定める。
      | 端子と接続　　　　　; 1 1 → MAIN_EN、2 2 → P_SHDN
      | 公称値の公差　　　　; ±1%（既存部品資料の値）
      | 部品資料の根拠　　　; Vishay D/CRCW e3データシート20035の抵抗値・注文型番構成との既存照合記録。実装後の熱・電圧適合とは別。
      | モデルの範囲　　　　; Simscape抵抗の集中定数表現。部品の許容差、定格電力、温度係数、寄生インダクタンスの適合を示すものではない。
      | モデル設定　　　　　; R=1 kΩ。これらは保存モデルの設定値であり、すべてが実部品の保証値という意味ではない。
      | 確認の範囲　　　　　; 本説明は保存回路の部品情報・端子割当・既存設計意図を整理したもの。今回の説明更新によって新たな動作試験や実機検証を実施した意味ではない。
      | 設計記録　　　　　　; evaluation\component_annotations_20261022_r01\before_graph.json
      | evaluation\component_annotations_20261022_r01\before_metadata.json
      | evaluation\protection_capacitor_integration_20261021_r01\final_delivery\independent_readback\physical_bom.json
      | evaluation\protection_capacitor_integration_20261021_r01\protection_review\component_net_map.json
      | 
      | 【この説明欄の略語・記号】
      | 用語1　　　　　　　 ; MCU：Microcontroller Unit（マイクロコントローラ）。プログラムを実行し、測定値の処理や出力制御を担当する小型計算機。
      | 用語2　　　　　　　 ; Hi-Z：High Impedance（高インピーダンス状態）。出力が強くHigh/Lowを駆動していない状態。プルアップやプルダウンによって端子電圧が決まる場合がある。
      | 用語3　　　　　　　 ; SHDN：Shutdown（停止制御端子）。LTC4364ではLowで停止を指示する。Highは動作許可であり、保護判定を無効にするものではない。
      | 用語4　　　　　　　 ; EN：Enable（動作許可）。対象機能の動作を許可する信号。端子ごとの有効レベルや接続状態に従う。
  R_FLT_PULLUP_10k : fl_lib/Electrical/Electrical Elements/Resistor  Description=|  R=22000 Ohm  i_specify=off  i_priority=None  i=0 A  i_nominal_specify=off  i_nominal_value=1  i_nominal_unit=A  v_specify=off  v_priority=None  v=0 V  v_nominal_specify=off  v_nominal_value=1  v_nominal_unit=V
      | この回路での名前　　; P_RFLT_PU
      | 部品名　　　　　　　; CRCW080522K0FKEA
      | この回路での役割　　; 保護IC LTC4364の故障通知を、マイコンがHigh・Lowとして読めるようにするための抵抗。
      | ここでの動き　　　　; ICが故障通知の出力を解放しているとき、22 kΩを通じて信号を3.3 VのHighへ引き上げる。故障通知を出すとIC自身がLowへ引き下げる。マイコン本体への給電ではなく、通知信号の電位を作る役目。
      | 
      | 【詳しい働き・仕様・接続・確認の範囲】
      | 部品種別　　　　　　; 故障通知プルアップ
      | 公称値　　　　　　　; 22 kΩ
      | 配置目的　　　　　　; LTC4364のオープンドレインFLTをMCUの3.3 V系へ引き上げる。
      | 意図する動作　　　　; 22 kΩ。FAULT時はICがLOWへ引き込む。現設計の通知名PROTECTION_FLT_NとP_FLT_Nは接続を介して同じ故障通知経路。
      | 端子と接続　　　　　; 1 1 → 3V3、2 2 → P_FLT_N
      | 公称値の公差　　　　; ±1%（既存部品資料の値）
      | 部品資料の根拠　　　; Vishay D/CRCW e3データシート20035の抵抗値・注文型番構成との既存照合記録。実装後の熱・電圧適合とは別。
      | モデルの範囲　　　　; Simscape抵抗の集中定数表現。部品の許容差、定格電力、温度係数、寄生インダクタンスの適合を示すものではない。
      | モデル設定　　　　　; R=22 kΩ。これらは保存モデルの設定値であり、すべてが実部品の保証値という意味ではない。
      | 確認の範囲　　　　　; 本説明は保存回路の部品情報・端子割当・既存設計意図を整理したもの。今回の説明更新によって新たな動作試験や実機検証を実施した意味ではない。
      | 設計記録　　　　　　; evaluation\component_annotations_20261022_r01\before_graph.json
      | evaluation\component_annotations_20261022_r01\before_metadata.json
      | evaluation\protection_capacitor_integration_20261021_r01\final_delivery\independent_readback\physical_bom.json
      | evaluation\protection_capacitor_integration_20261021_r01\protection_review\component_net_map.json
      | 
      | 【この説明欄の略語・記号】
      | 用語1　　　　　　　 ; IC：Integrated Circuit（集積回路）。複数の電子素子と機能を小さな半導体チップに集積した部品。
      | 用語2　　　　　　　 ; MCU：Microcontroller Unit（マイクロコントローラ）。プログラムを実行し、測定値の処理や出力制御を担当する小型計算機。
      | 用語3　　　　　　　 ; FLT：Fault（故障状態通知）。LTC4364の故障警告出力。全種類の異常や逆流を一律に通知する信号という意味ではない。
  R_SHDN_PULLDOWN_47k : fl_lib/Electrical/Electrical Elements/Resistor  Description=|  R=47000 Ohm  i_specify=off  i_priority=None  i=0 A  i_nominal_specify=off  i_nominal_value=1  i_nominal_unit=A  v_specify=off  v_priority=None  v=0 V  v_nominal_specify=off  v_nominal_value=1  v_nominal_unit=V
      | この回路での名前　　; P_RSHDN_PD
      | 部品名　　　　　　　; CRCW080547K0FKEA
      | この回路での役割　　; マイコンがまだ指令を出していない間、保護IC LTC4364を停止側に置くための抵抗。
      | ここでの動き　　　　; 動作許可・停止を受けるSHDN端子を47 kΩで共通GNDへ引き下げる。LTC4364内部には反対に引き上げる働きもあるので、実際に停止判定の電圧になるかはそれと合わせて確認する。
      | 
      | 【詳しい働き・仕様・接続・確認の範囲】
      | 部品種別　　　　　　; 停止制御入力プルダウン
      | 公称値　　　　　　　; 47 kΩ
      | 配置目的　　　　　　; SHDNをGNDへ下げ、MCU未駆動時に停止側へ保つ。
      | 意図する動作　　　　; LTC4364内部のSHDNプルアップも考慮する。接続の存在だけで全起動シーケンスの安全を保証しない。
      | 端子と接続　　　　　; 1 1 → P_SHDN、2 2 → GND
      | 公称値の公差　　　　; ±1%（既存部品資料の値）
      | 部品資料の根拠　　　; Vishay D/CRCW e3データシート20035の抵抗値・注文型番構成との既存照合記録。実装後の熱・電圧適合とは別。
      | モデルの範囲　　　　; Simscape抵抗の集中定数表現。部品の許容差、定格電力、温度係数、寄生インダクタンスの適合を示すものではない。
      | モデル設定　　　　　; R=47 kΩ。これらは保存モデルの設定値であり、すべてが実部品の保証値という意味ではない。
      | 確認の範囲　　　　　; 本説明は保存回路の部品情報・端子割当・既存設計意図を整理したもの。今回の説明更新によって新たな動作試験や実機検証を実施した意味ではない。
      | 設計記録　　　　　　; evaluation\component_annotations_20261022_r01\before_graph.json
      | evaluation\component_annotations_20261022_r01\before_metadata.json
      | evaluation\protection_capacitor_integration_20261021_r01\final_delivery\independent_readback\physical_bom.json
      | evaluation\protection_capacitor_integration_20261021_r01\protection_review\component_net_map.json
      | 
      | 【この説明欄の略語・記号】
      | 用語1　　　　　　　 ; MCU：Microcontroller Unit（マイクロコントローラ）。プログラムを実行し、測定値の処理や出力制御を担当する小型計算機。
      | 用語2　　　　　　　 ; GND：Ground（回路の基準電位・電流帰路）。この図の共通基準。保護接地や大地への接続を意味するとは限らない。
      | 用語3　　　　　　　 ; SHDN：Shutdown（停止制御端子）。LTC4364ではLowで停止を指示する。Highは動作許可であり、保護判定を無効にするものではない。
  SHDN_RETURN : ConnectionLabel  Description=|  Label=PROT_RETURN
      | この回路での名前　　; PROT_RETURN
      | 種別　　　　　　　　; ConnectionLabel
      | この回路での役割　　; 保護回路の帰路を、外側の共通GNDへ結ぶ。このラベルはプロトタイプという意味ではなく保護回路の戻り線を示す。明示的な境界端子を経由してBT1負極・PV1負極と同じノードになる。
      | 共通帰路の代表接続　; P_U1（保護MOSFETを制御する保護IC／LTC4364IMS-1#PBF）: GND
      |                     ; BT1（充電先の蓄電池／51.2V 100Ah LiFePO4）: -
      |                     ; PV1（直列太陽電池列の負極側パネル／400W panel 1/2）: -
      |                     ; U7（RP2040搭載Pico W／SC0918）: 3(GND), 8(GND), 13(GND), 18(GND), 23(GND), 28(GND), 33(AGND), 38(GND)
      |                     ; U1（外付けADC／MCP3208-CI/SL）: 8(CH7), 9(DGND), 14(AGND)
      | この場所の直接接続　; P_RSHDN_PD（SHDNをGNDへ下げ、MCU未駆動時に停止側へ保つ／47 kΩ）: 2
      | 直接接続の範囲　　　; このラベルから実際の線・分岐・明示的な境界端子だけを追った接続。同名ラベルによる離れた場所への接続はこの欄に含めない。
      | 同一ネット全端子　　; BT1: -
      |                     ; C1: 2(n)
      |                     ; C2: 2(n)
      |                     ; C3: 2(n)
      |                     ; C4: 2(n)
      |                     ; C7: 2(n)
      |                     ; C8: 2(n)
      |                     ; C9: 2(n)
      |                     ; C10: 2(n)
      |                     ; C13: 2(n)
      |                     ; C14: 2(n)
      |                     ; C15: 2(n)
      |                     ; C16: 2(n)
      |                     ; C17: 2
      |                     ; C18: 2
      |                     ; C19: 2
      |                     ; C20: 2
      |                     ; C21: 2
      |                     ; C22: 2
      |                     ; C23: 2
      |                     ; C24: 2
      |                     ; C25: 2
      |                     ; C26: 2
      |                     ; C27: 2
      |                     ; C28: 2
      |                     ; C29: 2
      |                     ; C30: 2
      |                     ; C31: 2
      |                     ; C33: 2
      |                     ; C34: 2
      |                     ; C35: 2
      |                     ; C36: 2
      |                     ; C40: 2
      |                     ; C41: 2
      |                     ; C42: 2
      |                     ; C43: 2
      |                     ; C44: 2
      |                     ; C45: 2
      |                     ; C46: 2
      |                     ; C47: 2
      |                     ; C48: 2
      |                     ; D2: 2(A)
      |                     ; PV1: -
      |                     ; P_CHG: N
      |                     ; P_COUT: N
      |                     ; P_CTMR: N
      |                     ; P_D1: A
      |                     ; P_R3: 2
      |                     ; P_R8: 2
      |                     ; P_RSHDN_PD: 2
      |                     ; P_U1: GND
      |                     ; Q2: 3(S)
      |                     ; Q3: 1(S1), 4(S2)
      |                     ; R1: 2(n)
      |                     ; R18: 2
      |                     ; R21: 2
      |                     ; R24: 2
      |                     ; R35: 2
      |                     ; R42: 2
      |                     ; R44: 2
      |                     ; R48: 2
      |                     ; U1: 8(CH7), 9(DGND), 14(AGND)
      |                     ; U2: 2(GND), 3(REF2), 4(RESERVED_GND)
      |                     ; U3: 2(GND), 3(REF2), 4(RESERVED_GND)
      |                     ; U4: 3(GND)
      |                     ; U5: 3(GND)
      |                     ; U6: 3(GND)
      |                     ; U7: 3(GND), 8(GND), 13(GND), 18(GND), 23(GND), 28(GND), 33(AGND), 38(GND)
      |                     ; U9: 4(VEE)
      |                     ; U10: 1(GNDP), 2(GNDP), 5(GNDP), 8(GNDP), 9(GNDP), 10(GNDP), 11(GNDP), 12(GNDP), 13(GNDP), 14(GNDP), 15(GNDP), 16(GNDP), 17(GNDP), 18(GNDP)
      |                     ; U11: 2(GND)
      |                     ; U12: 2(GND)
      | 接続部品数　　　　　; 72部品（部品番号で集計。同一ネット全体）
      | 接続端子数　　　　　; 99端子（423端子の部品対応表で集計。ラベル・境界ポートの重複は含めない）
      | この場所の端子数　　; 1端子／1部品（同名ラベルによる接続を除く）
      | 同階層同名ラベル数　; 8個（このラベル自身を含む）
      | 全階層の接続ラベル　; 87個（実際に同じノードへつながるラベル。名前が違う別名も含む）
      | 接続ルール　　　　　; 同じ階層の同じラベル名を仮想配線として結ぶ。別のSubsystem内とは名前だけでつながらず、明示的なConnection Portと配線をたどる。色は用途の表示であり接続を決めない。
      | 確認の範囲　　　　　; 現在の保存回路の端子・配線から求めた静的接続。抵抗やICの内部を導線として短絡せずに集計した。説明の更新は動作シミュレーション、タイミング、実部品の性能・実機動作を保証するものではない。
      | 記録の基準　　　　　; measurement_label_layout_20261022_r01/after_layout_graph.json。部品対応表は端子名の対応付けにのみ使用。
      | 
      | 【この説明欄の略語・記号】
      | 用語1　　　　　　　 ; ADC：Analog-to-Digital Converter（アナログ・デジタル変換器）。測定電圧をデジタル値へ変換する回路。電流や温度も、センサーで電圧へ変換した後に読み取る。
      | 用語2　　　　　　　 ; IC：Integrated Circuit（集積回路）。複数の電子素子と機能を小さな半導体チップに集積した部品。
      | 用語3　　　　　　　 ; MCU：Microcontroller Unit（マイクロコントローラ）。プログラムを実行し、測定値の処理や出力制御を担当する小型計算機。
      | 用語4　　　　　　　 ; CH：Channel（測定チャネル）。CH0〜CH7はADCの入力番号であり、同時測定を意味しない。
      | 用語5　　　　　　　 ; MOSFET：Metal-Oxide-Semiconductor Field-Effect Transistor（金属・酸化膜・半導体構造の電界効果トランジスタ）。ゲートとソースの電圧でドレインとソースの導通を制御する素子。N-MOSはNチャネル型を表す。
      | 用語6　　　　　　　 ; LiFePO4：Lithium Iron Phosphate（リン酸鉄リチウム）。電池の正極材料を示す化学式。英語の頭文字を並べた略語ではない。
      | 用語7　　　　　　　 ; GND：Ground（回路の基準電位・電流帰路）。この図の共通基準。保護接地や大地への接続を意味するとは限らない。
      | 用語8　　　　　　　 ; AGND：Analog Ground（アナログ回路の基準端子）。アナログ部分の電流帰路。現図では共通GNDへ接続されるが、実装時の電流経路への配慮は別途必要。
      | 用語9　　　　　　　 ; DGND：Digital Ground（デジタル回路の基準端子）。デジタル部分の電流帰路。現図では共通GNDへ接続される。
      | 用語10　　　　　　　; SHDN：Shutdown（停止制御端子）。LTC4364ではLowで停止を指示する。Highは動作許可であり、保護判定を無効にするものではない。
      | 用語11　　　　　　　; VREF/REF：基準電圧を表す端子名。REFはReference（基準）の意味。ADCの変換尺度や電流アンプの出力基準に使う。REF1/REF2の接続電位は個別に確認する。
      | 用語12　　　　　　　; VCC/VDD/VEE/VS：ICの電源端子名。文字の歴史的な由来を現在の接続機能へ当てはめない。現回路のVEEはU8/U10では浮動基準SW、U9ではGND。各電圧・基準は端子と接続を参照する。
      | 用語13　　　　　　　; GNDP：U10の一次側電源の基準端子。絶縁電源の入力側GND。二次側基準VEE=SWと直接同一の導体ではない。
      | 用語14　　　　　　　; SW：Switching Node（スイッチング点）。主電力段の上下MOSFETとL1がつながる、電圧が高速に切り替わる点。GNDとは別電位。
      | 用語15　　　　　　　; PROT_RETURN：保護回路の共通帰路。PROTはProtection（保護）、RETURNは帰路。プロトタイプの略ではなく、現回路では共通GNDへつながる。
  U1_LTC4364 : Subsystem  Description=|
      | この回路での名前　　; P_U1
      | 部品名　　　　　　　; LTC4364IMS-1#PBF
      | この回路での役割　　; 充電器と電池の間で、逆流を防ぎ、異常時には順方向の充電も制限・停止する保護IC。
      | ここでの動き　　　　; 外付けMOSFET P_Q1/P_Q2を動かして電流を通す・制限する・止める。設定した電圧や電流などを監視して独立に保護する。マイコンとの停止・故障通知の信号線は接続しているが、MicroPythonの制御との統合と一貫した動作試験は未完了。
      | 
      | 【詳しい働き・仕様・接続・確認の範囲】
      | 識別の補足　　　　　; P_U1（図上のブロック名：U1_LTC4364）
      | 部品名の補足　　　　; LTC4364IMS-1#PBF／Analog Devices（LTC4364-1、MSOP-16）
      | 詳しい役割　　　　　; 充電器と電池の間に置く保護IC。電池から充電器への逆流を防ぎ、異常時には充電器から電池へ流す順方向の給電も止める。実際に電流を通す・止めるのは、ICが駆動する外付けP_Q1/P_Q2。
      | 部品の分類　　　　　; Surge Stopper with Ideal Diode（サージストッパ＋理想ダイオード制御IC）。メーカーが一体化している機能の分類。
      | 通常時の動き　　　　; 充電器から電池へ電流を流す。P_Q1/P_Q2を通電させ、逆流防止をMOSFETで行うことでダイオードの順方向電圧降下による損失を抑える狙いがある。効率の改善量をここで保証するものではない。
      | 逆流時の動き　　　　; 電池側から充電器側へ電流が戻ろうとすると、DGATEでP_Q2をOFFへ制御して逆流を抑える。夜間など上流電圧が低下したときに、電池を上流へ放電させないための役割。
      | 異常時の動き　　　　; HGATEでP_Q1を制御し、出力の過電圧や過電流を制限する。設定した異常継続時間を超えると順方向の給電も停止する。採用する-1型は、この保護停止を保持するラッチ型であり、自動再試行型の-2とは異なる。
      | 独立保護の意味　　　; 通電が許可され、ICの動作条件が満たされている間は、保護判定をマイコンの計算に任せずICと周辺抵抗・コンデンサが行う。RP2040が通常の充電制御を担当し、このICが電力経路の保護を担当する。
      | マイコンとの関係　　; SHDN（採用MSOP-16品の9番端子）をLowにすると停止できる。Highは通電の許可であり、ICの保護判定を無効化する指令ではない。主電力段Q1/Q2へ送る相補PWMとは別のON/OFF制御。
      | 現在の接続　　　　　; RP2040のGP11 → MAIN_EN → MCU_EN → P_RSHDN_SER 1 kΩ → SHDNを接続済み。SHDNには47 kΩのプルダウンを置く。FLTは22 kΩで3.3 Vへプルアップし、PROTECTION_FLT_NからGP13へ接続する。
      | 現在の使用状態　　　; 独立保護回路をモデル化し、マイコン用の停止入力・故障通知の接続も用意済み。一方、現行c05用MicroPythonでの起動・停止・FLT監視・ラッチ復帰をまとめた統合実装と一貫試験は未完了。試験用GPIO刺激は、RP2040実行の確認とは区別する。
      | 拡張できること　　　; MicroPython側を追加・統合すれば、充電終了時の給電停止、測定値に応じた停止要求、故障の記録、原因解消を確認した後の復帰制御に利用できる。これは拡張候補であり、現状の完成済み機能とはしない。
      | 復帰時の注意　　　　; SHDNによるリセットも可能だが、原因が残ったまま繰り返し再投入しない。メーカーが示す冷却時間・リセット条件と、MOSFETの許容動作領域を確認して復帰シーケンスを決める。
      | 通知端子の意味　　　; FLTは保護タイマーに関係する異常予告・通知用のオープンドレイン出力であり、すべての異常や逆流を個別に知らせる信号ではない。ENOUTは現構成ではGPIO監視に未使用。
      | 端子と接続　　　　　; VCC VCC → P_VCC、HGATE HGATE → P_HGATE、SOURCE SOURCE → P_SOURCE、DGATE DGATE → P_DGATE、SENSE SENSE → P_SENSE、OUT OUT → BAT_PLUS、SHDN SHDN → P_SHDN、UV UV → P_UV、OV OV → P_OV、FB FB → P_FB、TMR TMR → P_TMR、GND GND → GND、FLT FLT → P_FLT_N、ENOUT ENOUT → P_ENOUT_UNUSED
      | メーカー資料　　　　; https://www.analog.com/media/en/technical-documentation/data-sheets/ltc4364-1-4364-2.pdf Rev.B：1頁の機能概要、8～9頁の端子説明、15頁の故障復帰条件、17頁のShutdown。
      | モデルの範囲　　　　; 内部IC_COREにプロジェクト作成のLTC4364機能近似モデルを置く。メーカーの認証済みSimscapeモデルではない。限定試験の結果と実部品の高速過渡・SOA・熱の適合を区別する。
      | 確認の範囲　　　　　; 本説明は保存回路の部品情報・端子割当・既存設計意図を整理したもの。今回の説明更新によって新たな動作試験や実機検証を実施した意味ではない。
      | 
      | 【この説明欄の略語・記号】
      | 用語1　　　　　　　 ; IC：Integrated Circuit（集積回路）。複数の電子素子と機能を小さな半導体チップに集積した部品。
      | 用語2　　　　　　　 ; MCU：Microcontroller Unit（マイクロコントローラ）。プログラムを実行し、測定値の処理や出力制御を担当する小型計算機。
      | 用語3　　　　　　　 ; PWM：Pulse Width Modulation（パルス幅変調）。周期に対するON時間の割合を変えて、スイッチの平均的な電力伝達を調整する方式。
      | 用語4　　　　　　　 ; GPIO：General-Purpose Input/Output（汎用入出力端子）。入力・出力や周辺機能に割り当てられる端子。GPの後の数字はRP2040の端子信号番号で、基板上の物理ピン番号とは別。
      | 用語5　　　　　　　 ; MOSFET：Metal-Oxide-Semiconductor Field-Effect Transistor（金属・酸化膜・半導体構造の電界効果トランジスタ）。ゲートとソースの電圧でドレインとソースの導通を制御する素子。N-MOSはNチャネル型を表す。
      | 用語6　　　　　　　 ; SOA：Safe Operating Area（安全動作領域）。素子が扱える電圧・電流・継続時間・温度の組合せ。耐圧や最大電流を個別に満たすだけではSOAの成立にならない。
      | 用語7　　　　　　　 ; MSOP：Mini Small Outline Package（小型の外形パッケージ形式）。末尾の16は端子数を表す。本部品ではMSOP-16の端子配置を使用する。
      | 用語8　　　　　　　 ; GND：Ground（回路の基準電位・電流帰路）。この図の共通基準。保護接地や大地への接続を意味するとは限らない。
      | 用語9　　　　　　　 ; SHDN：Shutdown（停止制御端子）。LTC4364ではLowで停止を指示する。Highは動作許可であり、保護判定を無効にするものではない。
      | 用語10　　　　　　　; FLT：Fault（故障状態通知）。LTC4364の故障警告出力。全種類の異常や逆流を一律に通知する信号という意味ではない。
      | 用語11　　　　　　　; UV：Undervoltage（低電圧検出）。LTC4364の入力電圧が低い状態を判定する端子。
      | 用語12　　　　　　　; OV：Overvoltage（過電圧検出）。LTC4364の入力側過電圧判定。FBで行う出力電圧制限とは機能が異なる。
      | 用語13　　　　　　　; FB：Feedback（帰還）。出力などを検出して内部制御へ戻すための信号・端子。
      | 用語14　　　　　　　; TMR：Timer（時間設定端子）。LTC4364では外付けコンデンサにより故障継続時間の判定などに関係する時間を設定する。
      | 用語15　　　　　　　; EN：Enable（動作許可）。対象機能の動作を許可する信号。端子ごとの有効レベルや接続状態に従う。
      | 用語16　　　　　　　; ENOUT：Enable Output（動作許可状態の出力）。LTC4364の下流回路向け許可出力。SHDNへの外部停止指示とは方向が逆の別端子。
      | 用語17　　　　　　　; VCC/VDD/VEE/VS：ICの電源端子名。文字の歴史的な由来を現在の接続機能へ当てはめない。現回路のVEEはU8/U10では浮動基準SW、U9ではGND。各電圧・基準は端子と接続を参照する。
      | 用語18　　　　　　　; HGATE/DGATE：LTC4364の二つの外付けMOSFETゲート駆動出力。HGATEは主に電圧・電流制限側のP_Q1、DGATEは理想ダイオード／逆流防止側のP_Q2を駆動する。主電力段の上下PWMとは別の仕組み。
      | 用語19　　　　　　　; SW：Switching Node（スイッチング点）。主電力段の上下MOSFETとL1がつながる、電圧が高速に切り替わる点。GNDとは別電位。
      | 
      | 
      | 【実物に対応する端子配置】
      | 表示の向き　　　　　; TOP VIEW / 1番端子が左上
      | 対象パッケージ　　　; MSOP-16
      | 番号の意味　　　　　; 図内の番号は実部品の端子番号。GPIO名やSimulink内部のポート番号とは区別する。未使用の端子にもメーカーの機能名を表示する。
      | 表示の範囲　　　　　; 端子の相対的な並びを示す。部品の寸法・縮尺や基板フットプリントを保証する図ではない。
      | メーカー根拠　　　　; https://www.analog.com/media/en/technical-documentation/data-sheets/ltc4364-1-4364-2.pdf
      mask Display:
      | color('black');
      | plot([0.005 0.995 0.995 0.005 0.005],[0.005 0.005 0.995 0.995 0.005]);
      | text(0.5,0.94,'P_U1','horizontalAlignment','center','texmode','off');
      | text(0.5,0.86,'TOP VIEW','horizontalAlignment','center','texmode','off');
      | plot([0.10 0.12 0.14 0.12 0.10],[0.97 0.99 0.97 0.95 0.97]);
      | port_label('lconn',1,'1 OUT');
      | port_label('lconn',2,'2 SENSE');
      | port_label('lconn',3,'3 NC');
      | port_label('lconn',4,'4 DGATE');
      | port_label('lconn',5,'5 SOURCE');
      | port_label('lconn',6,'6 HGATE');
      | port_label('lconn',7,'7 NC');
      | port_label('lconn',8,'8 VCC');
      | port_label('rconn',1,'16 FB');
      | port_label('rconn',2,'15 TMR');
      | port_label('rconn',3,'14 ENOUT');
      | port_label('rconn',4,'13 FLT');
      | port_label('rconn',5,'12 GND');
      | port_label('rconn',6,'11 OV');
      | port_label('rconn',7,'10 UV');
      | port_label('rconn',8,'9 SHDN');
  VIN : PMIOPort  Description=|  Side=Left
      | 識別名　　　　　　　; VIN
      | 種別　　　　　　　　; Simscape Connection Port（階層境界の物理端子）
      | 所属部品　　　　　　; LTC4364_Protection
      | 配置目的　　　　　　; 内部の電気ノードを、この外箱の外側の対応端子へ引き出す。
      | 対応端子　　　　　　; lconn:1
      | 接続ラベル　　　　　; VOUT
      | モデルの範囲　　　　; 実部品を1個追加する表現ではない。端子自体に増幅・遮断・測定機能を持たない。
      | 端子番号の注意　　　; Connection Portの番号は外箱内の対応番号であり、実パッケージのピン番号とは区別する。
      | 確認の範囲　　　　　; 実ポートと階層対応による静的接続の説明。電気特性の再現性は所属部品の説明を参照する。
      | 
      | 【この説明欄の略語・記号】
      | 用語1　　　　　　　 ; VIN/VOUT：入力電圧・出力電圧を表す端子／ネット名。INは入力、OUTは出力。電源変換器の電力端子なのか、検出用端子なのかは対象部品によって異なるため、端子と接続の説明に従う。
  VOUT : PMIOPort  Description=|  Port=2  Side=Right
      | 識別名　　　　　　　; VOUT
      | 種別　　　　　　　　; Simscape Connection Port（階層境界の物理端子）
      | 所属部品　　　　　　; LTC4364_Protection
      | 配置目的　　　　　　; 内部の電気ノードを、この外箱の外側の対応端子へ引き出す。
      | 対応端子　　　　　　; rconn:1
      | 接続ラベル　　　　　; BAT_PLUS
      | モデルの範囲　　　　; 実部品を1個追加する表現ではない。端子自体に増幅・遮断・測定機能を持たない。
      | 端子番号の注意　　　; Connection Portの番号は外箱内の対応番号であり、実パッケージのピン番号とは区別する。
      | 確認の範囲　　　　　; 実ポートと階層対応による静的接続の説明。電気特性の再現性は所属部品の説明を参照する。
      | 
      | 【この説明欄の略語・記号】
      | 用語1　　　　　　　 ; VIN/VOUT：入力電圧・出力電圧を表す端子／ネット名。INは入力、OUTは出力。電源変換器の電力端子なのか、検出用端子なのかは対象部品によって異なるため、端子と接続の説明に従う。
  MCU_EN : PMIOPort  Description=|  Port=3  Side=Left
      | 識別名　　　　　　　; MCU_EN
      | 種別　　　　　　　　; Simscape Connection Port（階層境界の物理端子）
      | 所属部品　　　　　　; LTC4364_Protection
      | 配置目的　　　　　　; 内部の電気ノードを、この外箱の外側の対応端子へ引き出す。
      | 対応端子　　　　　　; lconn:2
      | 接続ラベル　　　　　; MAIN_EN
      | モデルの範囲　　　　; 実部品を1個追加する表現ではない。端子自体に増幅・遮断・測定機能を持たない。
      | 端子番号の注意　　　; Connection Portの番号は外箱内の対応番号であり、実パッケージのピン番号とは区別する。
      | 確認の範囲　　　　　; 実ポートと階層対応による静的接続の説明。電気特性の再現性は所属部品の説明を参照する。
      | 
      | 【この説明欄の略語・記号】
      | 用語1　　　　　　　 ; MCU：Microcontroller Unit（マイクロコントローラ）。プログラムを実行し、測定値の処理や出力制御を担当する小型計算機。
      | 用語2　　　　　　　 ; EN：Enable（動作許可）。対象機能の動作を許可する信号。端子ごとの有効レベルや接続状態に従う。
  FLT : PMIOPort  Description=|  Port=4  Side=Right
      | 識別名　　　　　　　; FLT
      | 種別　　　　　　　　; Simscape Connection Port（階層境界の物理端子）
      | 所属部品　　　　　　; LTC4364_Protection
      | 配置目的　　　　　　; 内部の電気ノードを、この外箱の外側の対応端子へ引き出す。
      | 対応端子　　　　　　; rconn:2
      | 接続ラベル　　　　　; PROTECTION_FLT_N
      | モデルの範囲　　　　; 実部品を1個追加する表現ではない。端子自体に増幅・遮断・測定機能を持たない。
      | 端子番号の注意　　　; Connection Portの番号は外箱内の対応番号であり、実パッケージのピン番号とは区別する。
      | 確認の範囲　　　　　; 実ポートと階層対応による静的接続の説明。電気特性の再現性は所属部品の説明を参照する。
      | 
      | 【この説明欄の略語・記号】
      | 用語1　　　　　　　 ; FLT：Fault（故障状態通知）。LTC4364の故障警告出力。全種類の異常や逆流を一律に通知する信号という意味ではない。
  ENOUT : PMIOPort  Description=|  Port=5  Side=Right
      | 識別名　　　　　　　; ENOUT
      | 種別　　　　　　　　; Simscape Connection Port（階層境界の物理端子）
      | 所属部品　　　　　　; LTC4364_Protection
      | 配置目的　　　　　　; 内部の電気ノードを、この外箱の外側の対応端子へ引き出す。
      | 対応端子　　　　　　; rconn:3
      | 接続ラベル　　　　　; ラベルなし。接続は実線と境界対応で定義する。
      | モデルの範囲　　　　; 実部品を1個追加する表現ではない。端子自体に増幅・遮断・測定機能を持たない。
      | 端子番号の注意　　　; Connection Portの番号は外箱内の対応番号であり、実パッケージのピン番号とは区別する。
      | 確認の範囲　　　　　; 実ポートと階層対応による静的接続の説明。電気特性の再現性は所属部品の説明を参照する。
      | 
      | 【この説明欄の略語・記号】
      | 用語1　　　　　　　 ; SHDN：Shutdown（停止制御端子）。LTC4364ではLowで停止を指示する。Highは動作許可であり、保護判定を無効にするものではない。
      | 用語2　　　　　　　 ; ENOUT：Enable Output（動作許可状態の出力）。LTC4364の下流回路向け許可出力。SHDNへの外部停止指示とは方向が逆の別端子。
  RETURN : PMIOPort  Description=|  Port=6  Side=Left  ConnectionType=Connection: foundation.electrical.electrical
      | 識別名　　　　　　　; RETURN
      | 種別　　　　　　　　; Simscape Connection Port（階層境界の物理端子）
      | 所属部品　　　　　　; LTC4364_Protection
      | 配置目的　　　　　　; 内部の電気ノードを、この外箱の外側の対応端子へ引き出す。
      | 対応端子　　　　　　; lconn:3
      | 接続ラベル　　　　　; GND、PROT_RETURN
      | モデルの範囲　　　　; 実部品を1個追加する表現ではない。端子自体に増幅・遮断・測定機能を持たない。
      | 端子番号の注意　　　; Connection Portの番号は外箱内の対応番号であり、実パッケージのピン番号とは区別する。
      | 確認の範囲　　　　　; 実ポートと階層対応による静的接続の説明。電気特性の再現性は所属部品の説明を参照する。
      | 
      | 【この説明欄の略語・記号】
      | 用語1　　　　　　　 ; GND：Ground（回路の基準電位・電流帰路）。この図の共通基準。保護接地や大地への接続を意味するとは限らない。
      | 用語2　　　　　　　 ; PROT_RETURN：保護回路の共通帰路。PROTはProtection（保護）、RETURNは帰路。プロトタイプの略ではなく、現回路では共通GNDへつながる。
  VLOGIC : PMIOPort  Description=|  Port=7  Side=Left  ConnectionType=Connection: foundation.electrical.electrical
      | 識別名　　　　　　　; VLOGIC
      | 種別　　　　　　　　; Simscape Connection Port（階層境界の物理端子）
      | 所属部品　　　　　　; LTC4364_Protection
      | 配置目的　　　　　　; 内部の電気ノードを、この外箱の外側の対応端子へ引き出す。
      | 対応端子　　　　　　; lconn:4
      | 接続ラベル　　　　　; V3V3
      | モデルの範囲　　　　; 実部品を1個追加する表現ではない。端子自体に増幅・遮断・測定機能を持たない。
      | 端子番号の注意　　　; Connection Portの番号は外箱内の対応番号であり、実パッケージのピン番号とは区別する。
      | 確認の範囲　　　　　; 実ポートと階層対応による静的接続の説明。電気特性の再現性は所属部品の説明を参照する。
  connections:
  D6_Zener_15V/RConn1 -- CHG_47nF/LConn1 -- R5_10ohm/LConn1 -- U1_LTC4364/LConn6
  CHG_47nF/RConn1 -- RETURN_label_7/LConn1
  R7_226k/LConn1 -- COUT_330uF/LConn1 -- RSNS_10mOhm/RConn1 -- U1_LTC4364/LConn1 -- VOUT/RConn1
  COUT_330uF/RConn1 -- RETURN_label_4/LConn1
  CTMR_100nF/LConn1 -- U1_LTC4364/RConn2
  CTMR_100nF/RConn1 -- RETURN_label_5/LConn1
  D1_Zener_68V/LConn1 -- RETURN_label_6/LConn1
  R4_2k2/RConn1 -- D1_Zener_68V/RConn1 -- U1_LTC4364/LConn8
  D7_Zener_15V/LConn1 -- D6_Zener_15V/LConn1 -- M1_FDB33N25_APPROX/RConn2 -- M2_FDB3632_APPROX/RConn2 -- U1_LTC4364/LConn5
  M2_FDB3632_APPROX/LConn1 -- D7_Zener_15V/RConn1 -- U1_LTC4364/LConn4
  M1_FDB33N25_APPROX/LConn1 -- R5_10ohm/RConn1
  R1_205k/LConn1 -- M1_FDB33N25_APPROX/RConn1 -- R4_2k2/LConn1 -- VIN/RConn1
  RSNS_10mOhm/LConn1 -- M2_FDB3632_APPROX/RConn1 -- U1_LTC4364/LConn2
  R2_3k92/LConn1 -- R1_205k/RConn1 -- U1_LTC4364/RConn7
  R3_3k48/LConn1 -- R2_3k92/RConn1 -- U1_LTC4364/RConn6
  R3_3k48/RConn1 -- RETURN_label_2/LConn1
  R8_4k02/LConn1 -- R7_226k/RConn1 -- U1_LTC4364/RConn1
  R8_4k02/RConn1 -- RETURN_label_3/LConn1
  RETURN_label_1/LConn1 -- U1_LTC4364/RConn5
  R_EN_SERIES_1k/LConn1 -- MCU_EN/RConn1
  R_SHDN_PULLDOWN_47k/LConn1 -- R_EN_SERIES_1k/RConn1 -- U1_LTC4364/RConn8
  R_FLT_PULLUP_10k/LConn1 -- VLOGIC/RConn1
  U1_LTC4364/RConn4 -- R_FLT_PULLUP_10k/RConn1 -- FLT/RConn1
  SHDN_RETURN/LConn1 -- R_SHDN_PULLDOWN_47k/RConn1 -- RETURN/RConn1
  U1_LTC4364/RConn3 -- ENOUT/RConn1
